simulink model "rfsoc4x2_ospfb_128"  (R2021a)
settings: Solver=VariableStepAuto  StartTime=0.0  StopTime=2048  RelTol=1e-3
undefined symbols (not defined in the file): pfb_coeff_gen_calc
libraries: xbsIndex_r4 x37092, casper_library_delays x737, casper_library_misc x68, xps_library x1
(part 32 of 339)

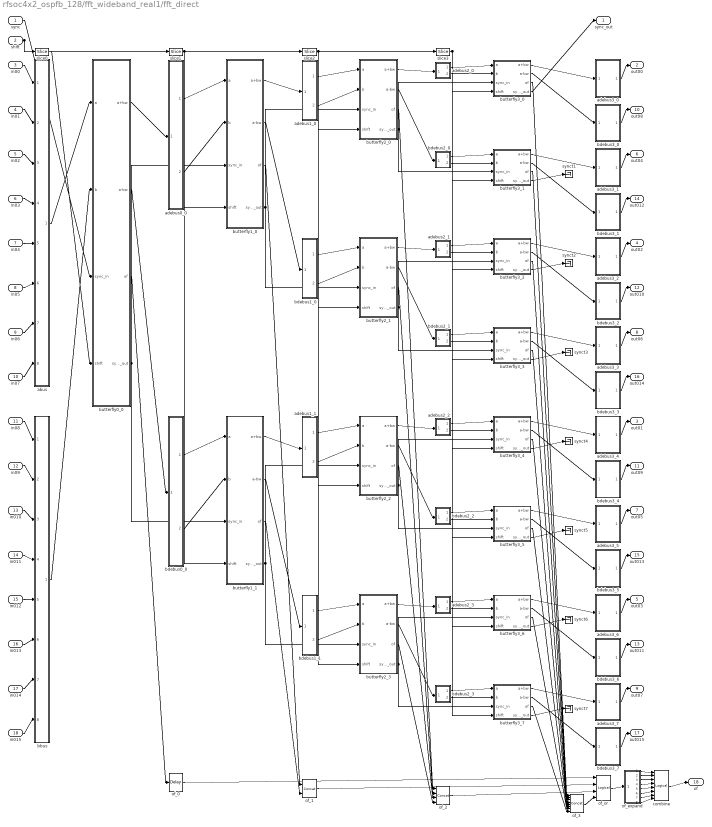
== system rfsoc4x2_ospfb_128/fft_wideband_real1/fft_direct ==
  sync : Inport
  shift : Inport  Port=2
  in00 : Inport  Port=3
  in01 : Inport  Port=4
  in02 : Inport  Port=5
  in03 : Inport  Port=6
  in04 : Inport  Port=7
  in05 : Inport  Port=8
  in06 : Inport  Port=9
  in07 : Inport  Port=10
  in08 : Inport  Port=11
  in09 : Inport  Port=12
  in010 : Inport  Port=13
  in011 : Inport  Port=14
  in012 : Inport  Port=15
  in013 : Inport  Port=16
  in014 : Inport  Port=17
  in015 : Inport  Port=18
  abus : Subsystem  AncestorBlock=casper_library_flow_control/bus_create  mask(bus_create){inputNum=8}
      mask prompts: inputNum "Number of inputs:"
      mask init:
      | bus_create_init(gcb,...
      |     'inputNum', inputNum);
  adebus0_0 : Subsystem  AncestorBlock=casper_library_flow_control/bus_expand  mask(bus_expand){mode=divisions of equal size, outputNum=2, outputWidth=[144 144], outputBinaryPt=[0 0], outputArithmeticType=[0 0], show_format=off, outputToWorkspace=off, variablePrefix=out, outputToModelAsWell=on}
      mask prompts: outputNum "Number of outputs:"; outputWidth "Output width:"; outputBinaryPt "Output binary point position:"; outputArithmeticType "Output arithmetic type (ufix=0, fix=1, bool=2):"; show_format "Print format string?"; outputToWorkspace "Output to workspace?"; variablePrefix "Variable name prefix:"; outputToModelAsWell "Output to model as well?"
      mask help:
      | Expands a 'bus' made using a bus_create or Xilinx
      | concat block.
      | The input will be divided into the specified number
      | of outputs with the specified arithmetic types.
      | Divisions are made from most significant bit.
      mask init: same as rfsoc4x2_ospfb_128/bus_expand1
      settings: AttributesFormatString=2 outputs
      mask TypeOptions mode: divisions of equal size | divisions of arbitrary size
      mask Callback mode: %bus_expand_callback();
      mask Callback outputWidth: %bus_expand_callback();
      mask Callback outputToWorkspace: %bus_expand_callback();
  adebus1_0 : Subsystem  AncestorBlock=casper_library_flow_control/bus_expand  mask(bus_expand){mode=divisions of equal size, outputNum=2, outputWidth=[72 72], outputBinaryPt=[0 0], outputArithmeticType=[0 0], show_format=off, outputToWorkspace=off, variablePrefix=out, outputToModelAsWell=on}
      mask prompts: outputNum "Number of outputs:"; outputWidth "Output width:"; outputBinaryPt "Output binary point position:"; outputArithmeticType "Output arithmetic type (ufix=0, fix=1, bool=2):"; show_format "Print format string?"; outputToWorkspace "Output to workspace?"; variablePrefix "Variable name prefix:"; outputToModelAsWell "Output to model as well?"
      mask help:
      | Expands a 'bus' made using a bus_create or Xilinx
      | concat block.
      | The input will be divided into the specified number
      | of outputs with the specified arithmetic types.
      | Divisions are made from most significant bit.
      mask init: same as rfsoc4x2_ospfb_128/bus_expand1
      settings: AttributesFormatString=2 outputs
      mask TypeOptions mode: divisions of equal size | divisions of arbitrary size
      mask Callback mode: %bus_expand_callback();
      mask Callback outputWidth: %bus_expand_callback();
      mask Callback outputToWorkspace: %bus_expand_callback();
  adebus1_1 : Subsystem  AncestorBlock=casper_library_flow_control/bus_expand  mask(bus_expand){mode=divisions of equal size, outputNum=2, outputWidth=[72 72], outputBinaryPt=[0 0], outputArithmeticType=[0 0], show_format=off, outputToWorkspace=off, variablePrefix=out, outputToModelAsWell=on}
      mask prompts: outputNum "Number of outputs:"; outputWidth "Output width:"; outputBinaryPt "Output binary point position:"; outputArithmeticType "Output arithmetic type (ufix=0, fix=1, bool=2):"; show_format "Print format string?"; outputToWorkspace "Output to workspace?"; variablePrefix "Variable name prefix:"; outputToModelAsWell "Output to model as well?"
      mask help:
      | Expands a 'bus' made using a bus_create or Xilinx
      | concat block.
      | The input will be divided into the specified number
      | of outputs with the specified arithmetic types.
      | Divisions are made from most significant bit.
      mask init: same as rfsoc4x2_ospfb_128/bus_expand1
      settings: AttributesFormatString=2 outputs
      mask TypeOptions mode: divisions of equal size | divisions of arbitrary size
      mask Callback mode: %bus_expand_callback();
      mask Callback outputWidth: %bus_expand_callback();
      mask Callback outputToWorkspace: %bus_expand_callback();
  adebus2_0 : Subsystem  AncestorBlock=casper_library_flow_control/bus_expand  mask(bus_expand){mode=divisions of equal size, outputNum=2, outputWidth=[36 36], outputBinaryPt=[0 0], outputArithmeticType=[0 0], show_format=off, outputToWorkspace=off, variablePrefix=out, outputToModelAsWell=on}
      mask prompts: outputNum "Number of outputs:"; outputWidth "Output width:"; outputBinaryPt "Output binary point position:"; outputArithmeticType "Output arithmetic type (ufix=0, fix=1, bool=2):"; show_format "Print format string?"; outputToWorkspace "Output to workspace?"; variablePrefix "Variable name prefix:"; outputToModelAsWell "Output to model as well?"
      mask help:
      | Expands a 'bus' made using a bus_create or Xilinx
      | concat block.
      | The input will be divided into the specified number
      | of outputs with the specified arithmetic types.
      | Divisions are made from most significant bit.
      mask init: same as rfsoc4x2_ospfb_128/bus_expand1
      settings: AttributesFormatString=2 outputs
      mask TypeOptions mode: divisions of equal size | divisions of arbitrary size
      mask Callback mode: %bus_expand_callback();
      mask Callback outputWidth: %bus_expand_callback();
      mask Callback outputToWorkspace: %bus_expand_callback();
  adebus2_1 : Subsystem  AncestorBlock=casper_library_flow_control/bus_expand  mask(bus_expand){mode=divisions of equal size, outputNum=2, outputWidth=[36 36], outputBinaryPt=[0 0], outputArithmeticType=[0 0], show_format=off, outputToWorkspace=off, variablePrefix=out, outputToModelAsWell=on}
      mask prompts: outputNum "Number of outputs:"; outputWidth "Output width:"; outputBinaryPt "Output binary point position:"; outputArithmeticType "Output arithmetic type (ufix=0, fix=1, bool=2):"; show_format "Print format string?"; outputToWorkspace "Output to workspace?"; variablePrefix "Variable name prefix:"; outputToModelAsWell "Output to model as well?"
      mask help:
      | Expands a 'bus' made using a bus_create or Xilinx
      | concat block.
      | The input will be divided into the specified number
      | of outputs with the specified arithmetic types.
      | Divisions are made from most significant bit.
      mask init: same as rfsoc4x2_ospfb_128/bus_expand1
      settings: AttributesFormatString=2 outputs
      mask TypeOptions mode: divisions of equal size | divisions of arbitrary size
      mask Callback mode: %bus_expand_callback();
      mask Callback outputWidth: %bus_expand_callback();
      mask Callback outputToWorkspace: %bus_expand_callback();
  adebus2_2 : Subsystem  AncestorBlock=casper_library_flow_control/bus_expand  mask(bus_expand){mode=divisions of equal size, outputNum=2, outputWidth=[36 36], outputBinaryPt=[0 0], outputArithmeticType=[0 0], show_format=off, outputToWorkspace=off, variablePrefix=out, outputToModelAsWell=on}
      mask prompts: outputNum "Number of outputs:"; outputWidth "Output width:"; outputBinaryPt "Output binary point position:"; outputArithmeticType "Output arithmetic type (ufix=0, fix=1, bool=2):"; show_format "Print format string?"; outputToWorkspace "Output to workspace?"; variablePrefix "Variable name prefix:"; outputToModelAsWell "Output to model as well?"
      mask help:
      | Expands a 'bus' made using a bus_create or Xilinx
      | concat block.
      | The input will be divided into the specified number
      | of outputs with the specified arithmetic types.
      | Divisions are made from most significant bit.
      mask init: same as rfsoc4x2_ospfb_128/bus_expand1
      settings: AttributesFormatString=2 outputs
      mask TypeOptions mode: divisions of equal size | divisions of arbitrary size
      mask Callback mode: %bus_expand_callback();
      mask Callback outputWidth: %bus_expand_callback();
      mask Callback outputToWorkspace: %bus_expand_callback();
  adebus2_3 : Subsystem  AncestorBlock=casper_library_flow_control/bus_expand  mask(bus_expand){mode=divisions of equal size, outputNum=2, outputWidth=[36 36], outputBinaryPt=[0 0], outputArithmeticType=[0 0], show_format=off, outputToWorkspace=off, variablePrefix=out, outputToModelAsWell=on}
      mask prompts: outputNum "Number of outputs:"; outputWidth "Output width:"; outputBinaryPt "Output binary point position:"; outputArithmeticType "Output arithmetic type (ufix=0, fix=1, bool=2):"; show_format "Print format string?"; outputToWorkspace "Output to workspace?"; variablePrefix "Variable name prefix:"; outputToModelAsWell "Output to model as well?"
      mask help:
      | Expands a 'bus' made using a bus_create or Xilinx
      | concat block.
      | The input will be divided into the specified number
      | of outputs with the specified arithmetic types.
      | Divisions are made from most significant bit.
      mask init: same as rfsoc4x2_ospfb_128/bus_expand1
      settings: AttributesFormatString=2 outputs
      mask TypeOptions mode: divisions of equal size | divisions of arbitrary size
      mask Callback mode: %bus_expand_callback();
      mask Callback outputWidth: %bus_expand_callback();
      mask Callback outputToWorkspace: %bus_expand_callback();
  adebus3_0 : Subsystem  AncestorBlock=casper_library_flow_control/bus_expand  mask(bus_expand){mode=divisions of equal size, outputNum=1, outputWidth=36, outputBinaryPt=0, outputArithmeticType=0, show_format=off, outputToWorkspace=off, variablePrefix=out, outputToModelAsWell=on}
      mask prompts: outputNum "Number of outputs:"; outputWidth "Output width:"; outputBinaryPt "Output binary point position:"; outputArithmeticType "Output arithmetic type (ufix=0, fix=1, bool=2):"; show_format "Print format string?"; outputToWorkspace "Output to workspace?"; variablePrefix "Variable name prefix:"; outputToModelAsWell "Output to model as well?"
      mask help:
      | Expands a 'bus' made using a bus_create or Xilinx
      | concat block.
      | The input will be divided into the specified number
      | of outputs with the specified arithmetic types.
      | Divisions are made from most significant bit.
      mask init: same as rfsoc4x2_ospfb_128/bus_expand1
      settings: AttributesFormatString=1 outputs
      mask TypeOptions mode: divisions of equal size | divisions of arbitrary size
      mask Callback mode: %bus_expand_callback();
      mask Callback outputWidth: %bus_expand_callback();
      mask Callback outputToWorkspace: %bus_expand_callback();
  adebus3_1 : Subsystem  AncestorBlock=casper_library_flow_control/bus_expand  mask(bus_expand){mode=divisions of equal size, outputNum=1, outputWidth=36, outputBinaryPt=0, outputArithmeticType=0, show_format=off, outputToWorkspace=off, variablePrefix=out, outputToModelAsWell=on}
      mask prompts: outputNum "Number of outputs:"; outputWidth "Output width:"; outputBinaryPt "Output binary point position:"; outputArithmeticType "Output arithmetic type (ufix=0, fix=1, bool=2):"; show_format "Print format string?"; outputToWorkspace "Output to workspace?"; variablePrefix "Variable name prefix:"; outputToModelAsWell "Output to model as well?"
      mask help:
      | Expands a 'bus' made using a bus_create or Xilinx
      | concat block.
      | The input will be divided into the specified number
      | of outputs with the specified arithmetic types.
      | Divisions are made from most significant bit.
      mask init: same as rfsoc4x2_ospfb_128/bus_expand1
      settings: AttributesFormatString=1 outputs
      mask TypeOptions mode: divisions of equal size | divisions of arbitrary size
      mask Callback mode: %bus_expand_callback();
      mask Callback outputWidth: %bus_expand_callback();
      mask Callback outputToWorkspace: %bus_expand_callback();
  adebus3_2 : Subsystem  AncestorBlock=casper_library_flow_control/bus_expand  mask(bus_expand){mode=divisions of equal size, outputNum=1, outputWidth=36, outputBinaryPt=0, outputArithmeticType=0, show_format=off, outputToWorkspace=off, variablePrefix=out, outputToModelAsWell=on}
      mask prompts: outputNum "Number of outputs:"; outputWidth "Output width:"; outputBinaryPt "Output binary point position:"; outputArithmeticType "Output arithmetic type (ufix=0, fix=1, bool=2):"; show_format "Print format string?"; outputToWorkspace "Output to workspace?"; variablePrefix "Variable name prefix:"; outputToModelAsWell "Output to model as well?"
      mask help:
      | Expands a 'bus' made using a bus_create or Xilinx
      | concat block.
      | The input will be divided into the specified number
      | of outputs with the specified arithmetic types.
      | Divisions are made from most significant bit.
      mask init: same as rfsoc4x2_ospfb_128/bus_expand1
      settings: AttributesFormatString=1 outputs
      mask TypeOptions mode: divisions of equal size | divisions of arbitrary size
      mask Callback mode: %bus_expand_callback();
      mask Callback outputWidth: %bus_expand_callback();
      mask Callback outputToWorkspace: %bus_expand_callback();
  adebus3_3 : Subsystem  AncestorBlock=casper_library_flow_control/bus_expand  mask(bus_expand){mode=divisions of equal size, outputNum=1, outputWidth=36, outputBinaryPt=0, outputArithmeticType=0, show_format=off, outputToWorkspace=off, variablePrefix=out, outputToModelAsWell=on}
      mask prompts: outputNum "Number of outputs:"; outputWidth "Output width:"; outputBinaryPt "Output binary point position:"; outputArithmeticType "Output arithmetic type (ufix=0, fix=1, bool=2):"; show_format "Print format string?"; outputToWorkspace "Output to workspace?"; variablePrefix "Variable name prefix:"; outputToModelAsWell "Output to model as well?"
      mask help:
      | Expands a 'bus' made using a bus_create or Xilinx
      | concat block.
      | The input will be divided into the specified number
      | of outputs with the specified arithmetic types.
      | Divisions are made from most significant bit.
      mask init: same as rfsoc4x2_ospfb_128/bus_expand1
      settings: AttributesFormatString=1 outputs
      mask TypeOptions mode: divisions of equal size | divisions of arbitrary size
      mask Callback mode: %bus_expand_callback();
      mask Callback outputWidth: %bus_expand_callback();
      mask Callback outputToWorkspace: %bus_expand_callback();
  adebus3_4 : Subsystem  AncestorBlock=casper_library_flow_control/bus_expand  mask(bus_expand){mode=divisions of equal size, outputNum=1, outputWidth=36, outputBinaryPt=0, outputArithmeticType=0, show_format=off, outputToWorkspace=off, variablePrefix=out, outputToModelAsWell=on}
      mask prompts: outputNum "Number of outputs:"; outputWidth "Output width:"; outputBinaryPt "Output binary point position:"; outputArithmeticType "Output arithmetic type (ufix=0, fix=1, bool=2):"; show_format "Print format string?"; outputToWorkspace "Output to workspace?"; variablePrefix "Variable name prefix:"; outputToModelAsWell "Output to model as well?"
      mask help:
      | Expands a 'bus' made using a bus_create or Xilinx
      | concat block.
      | The input will be divided into the specified number
      | of outputs with the specified arithmetic types.
      | Divisions are made from most significant bit.
      mask init: same as rfsoc4x2_ospfb_128/bus_expand1
      settings: AttributesFormatString=1 outputs
      mask TypeOptions mode: divisions of equal size | divisions of arbitrary size
      mask Callback mode: %bus_expand_callback();
      mask Callback outputWidth: %bus_expand_callback();
      mask Callback outputToWorkspace: %bus_expand_callback();
  adebus3_5 : Subsystem  AncestorBlock=casper_library_flow_control/bus_expand  mask(bus_expand){mode=divisions of equal size, outputNum=1, outputWidth=36, outputBinaryPt=0, outputArithmeticType=0, show_format=off, outputToWorkspace=off, variablePrefix=out, outputToModelAsWell=on}
      mask prompts: outputNum "Number of outputs:"; outputWidth "Output width:"; outputBinaryPt "Output binary point position:"; outputArithmeticType "Output arithmetic type (ufix=0, fix=1, bool=2):"; show_format "Print format string?"; outputToWorkspace "Output to workspace?"; variablePrefix "Variable name prefix:"; outputToModelAsWell "Output to model as well?"
      mask help:
      | Expands a 'bus' made using a bus_create or Xilinx
      | concat block.
      | The input will be divided into the specified number
      | of outputs with the specified arithmetic types.
      | Divisions are made from most significant bit.
      mask init: same as rfsoc4x2_ospfb_128/bus_expand1
      settings: AttributesFormatString=1 outputs
      mask TypeOptions mode: divisions of equal size | divisions of arbitrary size
      mask Callback mode: %bus_expand_callback();
      mask Callback outputWidth: %bus_expand_callback();
      mask Callback outputToWorkspace: %bus_expand_callback();
  adebus3_6 : Subsystem  AncestorBlock=casper_library_flow_control/bus_expand  mask(bus_expand){mode=divisions of equal size, outputNum=1, outputWidth=36, outputBinaryPt=0, outputArithmeticType=0, show_format=off, outputToWorkspace=off, variablePrefix=out, outputToModelAsWell=on}
      mask prompts: outputNum "Number of outputs:"; outputWidth "Output width:"; outputBinaryPt "Output binary point position:"; outputArithmeticType "Output arithmetic type (ufix=0, fix=1, bool=2):"; show_format "Print format string?"; outputToWorkspace "Output to workspace?"; variablePrefix "Variable name prefix:"; outputToModelAsWell "Output to model as well?"
      mask help:
      | Expands a 'bus' made using a bus_create or Xilinx
      | concat block.
      | The input will be divided into the specified number
      | of outputs with the specified arithmetic types.
      | Divisions are made from most significant bit.
      mask init: same as rfsoc4x2_ospfb_128/bus_expand1
      settings: AttributesFormatString=1 outputs
      mask TypeOptions mode: divisions of equal size | divisions of arbitrary size
      mask Callback mode: %bus_expand_callback();
      mask Callback outputWidth: %bus_expand_callback();
      mask Callback outputToWorkspace: %bus_expand_callback();
  adebus3_7 : Subsystem  AncestorBlock=casper_library_flow_control/bus_expand  mask(bus_expand){mode=divisions of equal size, outputNum=1, outputWidth=36, outputBinaryPt=0, outputArithmeticType=0, show_format=off, outputToWorkspace=off, variablePrefix=out, outputToModelAsWell=on}
      mask prompts: outputNum "Number of outputs:"; outputWidth "Output width:"; outputBinaryPt "Output binary point position:"; outputArithmeticType "Output arithmetic type (ufix=0, fix=1, bool=2):"; show_format "Print format string?"; outputToWorkspace "Output to workspace?"; variablePrefix "Variable name prefix:"; outputToModelAsWell "Output to model as well?"
      mask help:
      | Expands a 'bus' made using a bus_create or Xilinx
      | concat block.
      | The input will be divided into the specified number
      | of outputs with the specified arithmetic types.
      | Divisions are made from most significant bit.
      mask init: same as rfsoc4x2_ospfb_128/bus_expand1
      settings: AttributesFormatString=1 outputs
      mask TypeOptions mode: divisions of equal size | divisions of arbitrary size
      mask Callback mode: %bus_expand_callback();
      mask Callback outputWidth: %bus_expand_callback();
      mask Callback outputToWorkspace: %bus_expand_callback();
  bbus : Subsystem  AncestorBlock=casper_library_flow_control/bus_create  mask(bus_create){inputNum=8}
      mask prompts: inputNum "Number of inputs:"
      mask init:
      | bus_create_init(gcb,...
      |     'inputNum', inputNum);
  bdebus0_0 : Subsystem  AncestorBlock=casper_library_flow_control/bus_expand  mask(bus_expand){mode=divisions of equal size, outputNum=2, outputWidth=[144 144], outputBinaryPt=[0 0], outputArithmeticType=[0 0], show_format=off, outputToWorkspace=off, variablePrefix=out, outputToModelAsWell=on}
      mask prompts: outputNum "Number of outputs:"; outputWidth "Output width:"; outputBinaryPt "Output binary point position:"; outputArithmeticType "Output arithmetic type (ufix=0, fix=1, bool=2):"; show_format "Print format string?"; outputToWorkspace "Output to workspace?"; variablePrefix "Variable name prefix:"; outputToModelAsWell "Output to model as well?"
      mask help:
      | Expands a 'bus' made using a bus_create or Xilinx
      | concat block.
      | The input will be divided into the specified number
      | of outputs with the specified arithmetic types.
      | Divisions are made from most significant bit.
      mask init: same as rfsoc4x2_ospfb_128/bus_expand1
      settings: AttributesFormatString=2 outputs
      mask TypeOptions mode: divisions of equal size | divisions of arbitrary size
      mask Callback mode: %bus_expand_callback();
      mask Callback outputWidth: %bus_expand_callback();
      mask Callback outputToWorkspace: %bus_expand_callback();
  bdebus1_0 : Subsystem  AncestorBlock=casper_library_flow_control/bus_expand  mask(bus_expand){mode=divisions of equal size, outputNum=2, outputWidth=[72 72], outputBinaryPt=[0 0], outputArithmeticType=[0 0], show_format=off, outputToWorkspace=off, variablePrefix=out, outputToModelAsWell=on}
      mask prompts: outputNum "Number of outputs:"; outputWidth "Output width:"; outputBinaryPt "Output binary point position:"; outputArithmeticType "Output arithmetic type (ufix=0, fix=1, bool=2):"; show_format "Print format string?"; outputToWorkspace "Output to workspace?"; variablePrefix "Variable name prefix:"; outputToModelAsWell "Output to model as well?"
      mask help:
      | Expands a 'bus' made using a bus_create or Xilinx
      | concat block.
      | The input will be divided into the specified number
      | of outputs with the specified arithmetic types.
      | Divisions are made from most significant bit.
      mask init: same as rfsoc4x2_ospfb_128/bus_expand1
      settings: AttributesFormatString=2 outputs
      mask TypeOptions mode: divisions of equal size | divisions of arbitrary size
      mask Callback mode: %bus_expand_callback();
      mask Callback outputWidth: %bus_expand_callback();
      mask Callback outputToWorkspace: %bus_expand_callback();
  bdebus1_1 : Subsystem  AncestorBlock=casper_library_flow_control/bus_expand  mask(bus_expand){mode=divisions of equal size, outputNum=2, outputWidth=[72 72], outputBinaryPt=[0 0], outputArithmeticType=[0 0], show_format=off, outputToWorkspace=off, variablePrefix=out, outputToModelAsWell=on}
      mask prompts: outputNum "Number of outputs:"; outputWidth "Output width:"; outputBinaryPt "Output binary point position:"; outputArithmeticType "Output arithmetic type (ufix=0, fix=1, bool=2):"; show_format "Print format string?"; outputToWorkspace "Output to workspace?"; variablePrefix "Variable name prefix:"; outputToModelAsWell "Output to model as well?"
      mask help:
      | Expands a 'bus' made using a bus_create or Xilinx
      | concat block.
      | The input will be divided into the specified number
      | of outputs with the specified arithmetic types.
      | Divisions are made from most significant bit.
      mask init: same as rfsoc4x2_ospfb_128/bus_expand1
      settings: AttributesFormatString=2 outputs
      mask TypeOptions mode: divisions of equal size | divisions of arbitrary size
      mask Callback mode: %bus_expand_callback();
      mask Callback outputWidth: %bus_expand_callback();
      mask Callback outputToWorkspace: %bus_expand_callback();
  bdebus2_0 : Subsystem  AncestorBlock=casper_library_flow_control/bus_expand  mask(bus_expand){mode=divisions of equal size, outputNum=2, outputWidth=[36 36], outputBinaryPt=[0 0], outputArithmeticType=[0 0], show_format=off, outputToWorkspace=off, variablePrefix=out, outputToModelAsWell=on}
      mask prompts: outputNum "Number of outputs:"; outputWidth "Output width:"; outputBinaryPt "Output binary point position:"; outputArithmeticType "Output arithmetic type (ufix=0, fix=1, bool=2):"; show_format "Print format string?"; outputToWorkspace "Output to workspace?"; variablePrefix "Variable name prefix:"; outputToModelAsWell "Output to model as well?"
      mask help:
      | Expands a 'bus' made using a bus_create or Xilinx
      | concat block.
      | The input will be divided into the specified number
      | of outputs with the specified arithmetic types.
      | Divisions are made from most significant bit.
      mask init: same as rfsoc4x2_ospfb_128/bus_expand1
      settings: AttributesFormatString=2 outputs
      mask TypeOptions mode: divisions of equal size | divisions of arbitrary size
      mask Callback mode: %bus_expand_callback();
      mask Callback outputWidth: %bus_expand_callback();
      mask Callback outputToWorkspace: %bus_expand_callback();
  bdebus2_1 : Subsystem  AncestorBlock=casper_library_flow_control/bus_expand  mask(bus_expand){mode=divisions of equal size, outputNum=2, outputWidth=[36 36], outputBinaryPt=[0 0], outputArithmeticType=[0 0], show_format=off, outputToWorkspace=off, variablePrefix=out, outputToModelAsWell=on}
      mask prompts: outputNum "Number of outputs:"; outputWidth "Output width:"; outputBinaryPt "Output binary point position:"; outputArithmeticType "Output arithmetic type (ufix=0, fix=1, bool=2):"; show_format "Print format string?"; outputToWorkspace "Output to workspace?"; variablePrefix "Variable name prefix:"; outputToModelAsWell "Output to model as well?"
      mask help:
      | Expands a 'bus' made using a bus_create or Xilinx
      | concat block.
      | The input will be divided into the specified number
      | of outputs with the specified arithmetic types.
      | Divisions are made from most significant bit.
      mask init: same as rfsoc4x2_ospfb_128/bus_expand1
      settings: AttributesFormatString=2 outputs
      mask TypeOptions mode: divisions of equal size | divisions of arbitrary size
      mask Callback mode: %bus_expand_callback();
      mask Callback outputWidth: %bus_expand_callback();
      mask Callback outputToWorkspace: %bus_expand_callback();
  bdebus2_2 : Subsystem  AncestorBlock=casper_library_flow_control/bus_expand  mask(bus_expand){mode=divisions of equal size, outputNum=2, outputWidth=[36 36], outputBinaryPt=[0 0], outputArithmeticType=[0 0], show_format=off, outputToWorkspace=off, variablePrefix=out, outputToModelAsWell=on}
      mask prompts: outputNum "Number of outputs:"; outputWidth "Output width:"; outputBinaryPt "Output binary point position:"; outputArithmeticType "Output arithmetic type (ufix=0, fix=1, bool=2):"; show_format "Print format string?"; outputToWorkspace "Output to workspace?"; variablePrefix "Variable name prefix:"; outputToModelAsWell "Output to model as well?"
      mask help:
      | Expands a 'bus' made using a bus_create or Xilinx
      | concat block.
      | The input will be divided into the specified number
      | of outputs with the specified arithmetic types.
      | Divisions are made from most significant bit.
      mask init: same as rfsoc4x2_ospfb_128/bus_expand1
      settings: AttributesFormatString=2 outputs
      mask TypeOptions mode: divisions of equal size | divisions of arbitrary size
      mask Callback mode: %bus_expand_callback();
      mask Callback outputWidth: %bus_expand_callback();
      mask Callback outputToWorkspace: %bus_expand_callback();
  bdebus2_3 : Subsystem  AncestorBlock=casper_library_flow_control/bus_expand  mask(bus_expand){mode=divisions of equal size, outputNum=2, outputWidth=[36 36], outputBinaryPt=[0 0], outputArithmeticType=[0 0], show_format=off, outputToWorkspace=off, variablePrefix=out, outputToModelAsWell=on}
      mask prompts: outputNum "Number of outputs:"; outputWidth "Output width:"; outputBinaryPt "Output binary point position:"; outputArithmeticType "Output arithmetic type (ufix=0, fix=1, bool=2):"; show_format "Print format string?"; outputToWorkspace "Output to workspace?"; variablePrefix "Variable name prefix:"; outputToModelAsWell "Output to model as well?"
      mask help:
      | Expands a 'bus' made using a bus_create or Xilinx
      | concat block.
      | The input will be divided into the specified number
      | of outputs with the specified arithmetic types.
      | Divisions are made from most significant bit.
      mask init: same as rfsoc4x2_ospfb_128/bus_expand1
      settings: AttributesFormatString=2 outputs
      mask TypeOptions mode: divisions of equal size | divisions of arbitrary size
      mask Callback mode: %bus_expand_callback();
      mask Callback outputWidth: %bus_expand_callback();
      mask Callback outputToWorkspace: %bus_expand_callback();
  bdebus3_0 : Subsystem  AncestorBlock=casper_library_flow_control/bus_expand  mask(bus_expand){mode=divisions of equal size, outputNum=1, outputWidth=36, outputBinaryPt=0, outputArithmeticType=0, show_format=off, outputToWorkspace=off, variablePrefix=out, outputToModelAsWell=on}
      mask prompts: outputNum "Number of outputs:"; outputWidth "Output width:"; outputBinaryPt "Output binary point position:"; outputArithmeticType "Output arithmetic type (ufix=0, fix=1, bool=2):"; show_format "Print format string?"; outputToWorkspace "Output to workspace?"; variablePrefix "Variable name prefix:"; outputToModelAsWell "Output to model as well?"
      mask help:
      | Expands a 'bus' made using a bus_create or Xilinx
      | concat block.
      | The input will be divided into the specified number
      | of outputs with the specified arithmetic types.
      | Divisions are made from most significant bit.
      mask init: same as rfsoc4x2_ospfb_128/bus_expand1
      settings: AttributesFormatString=1 outputs
      mask TypeOptions mode: divisions of equal size | divisions of arbitrary size
      mask Callback mode: %bus_expand_callback();
      mask Callback outputWidth: %bus_expand_callback();
      mask Callback outputToWorkspace: %bus_expand_callback();
  bdebus3_1 : Subsystem  AncestorBlock=casper_library_flow_control/bus_expand  mask(bus_expand){mode=divisions of equal size, outputNum=1, outputWidth=36, outputBinaryPt=0, outputArithmeticType=0, show_format=off, outputToWorkspace=off, variablePrefix=out, outputToModelAsWell=on}
      mask prompts: outputNum "Number of outputs:"; outputWidth "Output width:"; outputBinaryPt "Output binary point position:"; outputArithmeticType "Output arithmetic type (ufix=0, fix=1, bool=2):"; show_format "Print format string?"; outputToWorkspace "Output to workspace?"; variablePrefix "Variable name prefix:"; outputToModelAsWell "Output to model as well?"
      mask help:
      | Expands a 'bus' made using a bus_create or Xilinx
      | concat block.
      | The input will be divided into the specified number
      | of outputs with the specified arithmetic types.
      | Divisions are made from most significant bit.
      mask init: same as rfsoc4x2_ospfb_128/bus_expand1
      settings: AttributesFormatString=1 outputs
      mask TypeOptions mode: divisions of equal size | divisions of arbitrary size
      mask Callback mode: %bus_expand_callback();
      mask Callback outputWidth: %bus_expand_callback();
      mask Callback outputToWorkspace: %bus_expand_callback();
  bdebus3_2 : Subsystem  AncestorBlock=casper_library_flow_control/bus_expand  mask(bus_expand){mode=divisions of equal size, outputNum=1, outputWidth=36, outputBinaryPt=0, outputArithmeticType=0, show_format=off, outputToWorkspace=off, variablePrefix=out, outputToModelAsWell=on}
      mask prompts: outputNum "Number of outputs:"; outputWidth "Output width:"; outputBinaryPt "Output binary point position:"; outputArithmeticType "Output arithmetic type (ufix=0, fix=1, bool=2):"; show_format "Print format string?"; outputToWorkspace "Output to workspace?"; variablePrefix "Variable name prefix:"; outputToModelAsWell "Output to model as well?"
      mask help:
      | Expands a 'bus' made using a bus_create or Xilinx
      | concat block.
      | The input will be divided into the specified number
      | of outputs with the specified arithmetic types.
      | Divisions are made from most significant bit.
      mask init: same as rfsoc4x2_ospfb_128/bus_expand1
      settings: AttributesFormatString=1 outputs
      mask TypeOptions mode: divisions of equal size | divisions of arbitrary size
      mask Callback mode: %bus_expand_callback();
      mask Callback outputWidth: %bus_expand_callback();
      mask Callback outputToWorkspace: %bus_expand_callback();
  bdebus3_3 : Subsystem  AncestorBlock=casper_library_flow_control/bus_expand  mask(bus_expand){mode=divisions of equal size, outputNum=1, outputWidth=36, outputBinaryPt=0, outputArithmeticType=0, show_format=off, outputToWorkspace=off, variablePrefix=out, outputToModelAsWell=on}
      mask prompts: outputNum "Number of outputs:"; outputWidth "Output width:"; outputBinaryPt "Output binary point position:"; outputArithmeticType "Output arithmetic type (ufix=0, fix=1, bool=2):"; show_format "Print format string?"; outputToWorkspace "Output to workspace?"; variablePrefix "Variable name prefix:"; outputToModelAsWell "Output to model as well?"
      mask help:
      | Expands a 'bus' made using a bus_create or Xilinx
      | concat block.
      | The input will be divided into the specified number
      | of outputs with the specified arithmetic types.
      | Divisions are made from most significant bit.
      mask init: same as rfsoc4x2_ospfb_128/bus_expand1
      settings: AttributesFormatString=1 outputs
      mask TypeOptions mode: divisions of equal size | divisions of arbitrary size
      mask Callback mode: %bus_expand_callback();
      mask Callback outputWidth: %bus_expand_callback();
      mask Callback outputToWorkspace: %bus_expand_callback();
  bdebus3_4 : Subsystem  AncestorBlock=casper_library_flow_control/bus_expand  mask(bus_expand){mode=divisions of equal size, outputNum=1, outputWidth=36, outputBinaryPt=0, outputArithmeticType=0, show_format=off, outputToWorkspace=off, variablePrefix=out, outputToModelAsWell=on}
      mask prompts: outputNum "Number of outputs:"; outputWidth "Output width:"; outputBinaryPt "Output binary point position:"; outputArithmeticType "Output arithmetic type (ufix=0, fix=1, bool=2):"; show_format "Print format string?"; outputToWorkspace "Output to workspace?"; variablePrefix "Variable name prefix:"; outputToModelAsWell "Output to model as well?"
      mask help:
      | Expands a 'bus' made using a bus_create or Xilinx
      | concat block.
      | The input will be divided into the specified number
      | of outputs with the specified arithmetic types.
      | Divisions are made from most significant bit.
      mask init: same as rfsoc4x2_ospfb_128/bus_expand1
      settings: AttributesFormatString=1 outputs
      mask TypeOptions mode: divisions of equal size | divisions of arbitrary size
      mask Callback mode: %bus_expand_callback();
      mask Callback outputWidth: %bus_expand_callback();
      mask Callback outputToWorkspace: %bus_expand_callback();
  bdebus3_5 : Subsystem  AncestorBlock=casper_library_flow_control/bus_expand  mask(bus_expand){mode=divisions of equal size, outputNum=1, outputWidth=36, outputBinaryPt=0, outputArithmeticType=0, show_format=off, outputToWorkspace=off, variablePrefix=out, outputToModelAsWell=on}
      mask prompts: outputNum "Number of outputs:"; outputWidth "Output width:"; outputBinaryPt "Output binary point position:"; outputArithmeticType "Output arithmetic type (ufix=0, fix=1, bool=2):"; show_format "Print format string?"; outputToWorkspace "Output to workspace?"; variablePrefix "Variable name prefix:"; outputToModelAsWell "Output to model as well?"
      mask help:
      | Expands a 'bus' made using a bus_create or Xilinx
      | concat block.
      | The input will be divided into the specified number
      | of outputs with the specified arithmetic types.
      | Divisions are made from most significant bit.
      mask init: same as rfsoc4x2_ospfb_128/bus_expand1
      settings: AttributesFormatString=1 outputs
      mask TypeOptions mode: divisions of equal size | divisions of arbitrary size
      mask Callback mode: %bus_expand_callback();
      mask Callback outputWidth: %bus_expand_callback();
      mask Callback outputToWorkspace: %bus_expand_callback();
  bdebus3_6 : Subsystem  AncestorBlock=casper_library_flow_control/bus_expand  mask(bus_expand){mode=divisions of equal size, outputNum=1, outputWidth=36, outputBinaryPt=0, outputArithmeticType=0, show_format=off, outputToWorkspace=off, variablePrefix=out, outputToModelAsWell=on}
      mask prompts: outputNum "Number of outputs:"; outputWidth "Output width:"; outputBinaryPt "Output binary point position:"; outputArithmeticType "Output arithmetic type (ufix=0, fix=1, bool=2):"; show_format "Print format string?"; outputToWorkspace "Output to workspace?"; variablePrefix "Variable name prefix:"; outputToModelAsWell "Output to model as well?"
      mask help:
      | Expands a 'bus' made using a bus_create or Xilinx
      | concat block.
      | The input will be divided into the specified number
      | of outputs with the specified arithmetic types.
      | Divisions are made from most significant bit.
      mask init: same as rfsoc4x2_ospfb_128/bus_expand1
      settings: AttributesFormatString=1 outputs
      mask TypeOptions mode: divisions of equal size | divisions of arbitrary size
      mask Callback mode: %bus_expand_callback();
      mask Callback outputWidth: %bus_expand_callback();
      mask Callback outputToWorkspace: %bus_expand_callback();
  bdebus3_7 : Subsystem  AncestorBlock=casper_library_flow_control/bus_expand  mask(bus_expand){mode=divisions of equal size, outputNum=1, outputWidth=36, outputBinaryPt=0, outputArithmeticType=0, show_format=off, outputToWorkspace=off, variablePrefix=out, outputToModelAsWell=on}
      mask prompts: outputNum "Number of outputs:"; outputWidth "Output width:"; outputBinaryPt "Output binary point position:"; outputArithmeticType "Output arithmetic type (ufix=0, fix=1, bool=2):"; show_format "Print format string?"; outputToWorkspace "Output to workspace?"; variablePrefix "Variable name prefix:"; outputToModelAsWell "Output to model as well?"
      mask help:
      | Expands a 'bus' made using a bus_create or Xilinx
      | concat block.
      | The input will be divided into the specified number
      | of outputs with the specified arithmetic types.
      | Divisions are made from most significant bit.
      mask init: same as rfsoc4x2_ospfb_128/bus_expand1
      settings: AttributesFormatString=1 outputs
      mask TypeOptions mode: divisions of equal size | divisions of arbitrary size
      mask Callback mode: %bus_expand_callback();
      mask Callback outputWidth: %bus_expand_callback();
      mask Callback outputToWorkspace: %bus_expand_callback();
  butterfly0_0 : Subsystem  AncestorBlock=casper_library_ffts/butterfly_direct  mask(butterfly_direct){n_inputs=8, biplex=off, FFTSize=8, Coeffs=[ 0 8 4 12 2 10 6 14 1 9 5 13 3 11 7 15], StepPeriod=0, coeff_bit_width=18, input_bit_width=18, bin_pt_in=17, downshift=off, async=off, floating_point=off, float_type=single, exp_width=8, frac_width=24, add_latency=1, mult_latency=3, bram_latency=3, conv_latency=3, add_pipe_latency=0, mult_pipe_latency=0, quantization=Round  (unbiased: +/- Inf), overflow=Wrap, coeffs_bit_limit=8, coeff_sharing=off, coeff_decimation=off, coeff_generation=off, cal_bits=1, n_bits_rotation=25, max_fanout=4, use_hdl=on, use_embedded=off, bitgrowth=off, hardcode_shifts=off, dsp48_adders=off}
      mask prompts: n_inputs "number inputs"; biplex "Used in biplex FFT"; FFTSize "Size of FFT: (2^? pts)"; Coeffs "Coefficients: (0 to 2^(FFTSize-1)-1)"; StepPeriod "Coefficient Step Period: (2^?)"; coeff_bit_width "Coefficient Bit Width"; input_bit_width "Input Bit Width"; bin_pt_in "Input binary point"; async "asynchronous operation"; floating_point "floating point"; float_type "float type"; exp_width "exponent width"; frac_width "fraction width"; add_latency "Add Latency"; mult_latency "Mult Latency"; bram_latency "BRAM Latency"; conv_latency "Convert latency"; add_pipe_latency "Add Pipeline Latency"; mult_pipe_latency "Mult Pipeline Latency"; quantization "Quantization Behavior"; overflow "Overflow Behavior"; coeffs_bit_limit "Number bits above which to store stage's coefficients in BRAM (2^? bits)"; coeff_sharing "BRAM sharing in coeff storage"; coeff_decimation "Store a fraction of coeff factors where useful"; coeff_generation "Generate coeffs with multipliers where useful"; cal_bits "Number calibration locations when generating coeffs (2^?)"; n_bits_rotation "Feedback rotation vector resolution"; max_fanout "Maximum fanout"; use_hdl "Use behavioural HDL for multipliers"; use_embedded "Use embedded multipliers"; bitgrowth "Bit growth instead of shifting"; hardcode_shifts "Hardcode shift schedule"; dsp48_adders "Use DSP48s for adders"
      mask help: FFT internal block.
      mask init: same as rfsoc4x2_ospfb_128/fft2/fft_direct/butterfly0_0
      settings: AttributesFormatString=twiddle_general
      mask Callback floating_point:
      | onoff = get_param(gcb, 'floating_point');
      | if strcmp(onoff,'on')
      |     enable_fixpt = 'off';
      |     set_param_state(gcb, 'float_type', 'on')
      | 
      |     f_type = get_param(gcb, 'float_type');
      |     if strcmp(f_type,'custom')
      |         set_param_state(gcb, 'exp_width', 'on')
      |         set_param_state(gcb, 'frac_width', 'on')
      |     else
      |         set_param_state(gcb, 'exp_width', 'off')
      |         set_param_state(gcb, 'frac_width', 'off')
      |     end
      | 
      | 
      | else
      |     enable_fixpt = 'on';
      |     set_param_state(gcb, 'float_type', 'off')
      |     set_param_state(gcb, 'exp_width', 'off')
      |     set_param_state(gcb, 'frac_width', 'off')
      | end
      | 
      | set_param_state(gcb, 'input_bit_width', enable_fixpt)
      | set_param_state(gcb, 'bin_pt_in', enable_fixpt)
      | set_param_state(gcb, 'coeff_bit_width', enable_fixpt)
      mask TypeOptions float_type: single | custom
      mask Callback float_type:
      | f_type = get_param(gcb, 'float_type');
      | if strcmp(f_type,'custom')
      |     set_param_state(gcb, 'exp_width', 'on')
      |     set_param_state(gcb, 'frac_width', 'on')
      | else
      |     set_param_state(gcb, 'exp_width', 'off')
      |     set_param_state(gcb, 'frac_width', 'off')
      | end
      mask TypeOptions quantization: Truncate | Round  (unbiased: +/- Inf) | Round  (unbiased: Even Values)
      mask TypeOptions overflow: Wrap | Saturate | Error
      mask Callback use_hdl:
      | % make mutually exclusive with use_embedded.
      | 
      | use_hdl = get_param(gcb, 'use_hdl');
      | if strcmp(use_hdl, 'on'),
      |     set_param_state(gcb, 'use_embedded', 'off');
      | else
      |     set_param_state(gcb, 'use_embedded', 'on');
      | end
      mask Callback use_embedded:
      | % make mutually exclusive with use_hdl.
      | 
      | use_hdl = get_param(gcb, 'use_embedded');
      | if strcmp(use_hdl, 'on'),
      |     set_param_state(gcb, 'use_hdl', 'off');
      | else
      |     set_param_state(gcb, 'use_hdl', 'on');
      | end
      mask Callback hardcode_shifts:
      | hardcode_shifts = get_param(gcb, 'hardcode_shifts');
      | set_param_state(gcb, 'downshift', hardcode_shifts);
      mask Callback dsp48_adders: %fft_callback_dsp48_adders(gcb);
      mask DialogControl ParameterTabVar0 Prompt: Basic
      mask DialogControl ParameterTabVar01 Prompt: Latency
      mask DialogControl ParameterTabVar012 Prompt: Implementation
  butterfly1_0 : Subsystem  AncestorBlock=casper_library_ffts/butterfly_direct  mask(butterfly_direct){n_inputs=4, biplex=off, FFTSize=8, Coeffs=[ 0 16 8 24 4 20 12 28 2 18 10 26 6 22 14 30], StepPeriod=0, coeff_bit_width=18, input_bit_width=18, bin_pt_in=17, downshift=off, async=off, floating_point=off, float_type=single, exp_width=8, frac_width=24, add_latency=1, mult_latency=3, bram_latency=3, conv_latency=3, add_pipe_latency=0, mult_pipe_latency=0, quantization=Round  (unbiased: +/- Inf), overflow=Wrap, coeffs_bit_limit=8, coeff_sharing=off, coeff_decimation=off, coeff_generation=off, cal_bits=1, n_bits_rotation=25, max_fanout=4, use_hdl=on, use_embedded=off, bitgrowth=off, hardcode_shifts=off, dsp48_adders=off}
      mask prompts: n_inputs "number inputs"; biplex "Used in biplex FFT"; FFTSize "Size of FFT: (2^? pts)"; Coeffs "Coefficients: (0 to 2^(FFTSize-1)-1)"; StepPeriod "Coefficient Step Period: (2^?)"; coeff_bit_width "Coefficient Bit Width"; input_bit_width "Input Bit Width"; bin_pt_in "Input binary point"; async "asynchronous operation"; floating_point "floating point"; float_type "float type"; exp_width "exponent width"; frac_width "fraction width"; add_latency "Add Latency"; mult_latency "Mult Latency"; bram_latency "BRAM Latency"; conv_latency "Convert latency"; add_pipe_latency "Add Pipeline Latency"; mult_pipe_latency "Mult Pipeline Latency"; quantization "Quantization Behavior"; overflow "Overflow Behavior"; coeffs_bit_limit "Number bits above which to store stage's coefficients in BRAM (2^? bits)"; coeff_sharing "BRAM sharing in coeff storage"; coeff_decimation "Store a fraction of coeff factors where useful"; coeff_generation "Generate coeffs with multipliers where useful"; cal_bits "Number calibration locations when generating coeffs (2^?)"; n_bits_rotation "Feedback rotation vector resolution"; max_fanout "Maximum fanout"; use_hdl "Use behavioural HDL for multipliers"; use_embedded "Use embedded multipliers"; bitgrowth "Bit growth instead of shifting"; hardcode_shifts "Hardcode shift schedule"; dsp48_adders "Use DSP48s for adders"
      mask help: FFT internal block.
      mask init: same as rfsoc4x2_ospfb_128/fft2/fft_direct/butterfly0_0
      settings: AttributesFormatString=twiddle_general
      mask Callback floating_point:
      | onoff = get_param(gcb, 'floating_point');
      | if strcmp(onoff,'on')
      |     enable_fixpt = 'off';
      |     set_param_state(gcb, 'float_type', 'on')
      | 
      |     f_type = get_param(gcb, 'float_type');
      |     if strcmp(f_type,'custom')
      |         set_param_state(gcb, 'exp_width', 'on')
      |         set_param_state(gcb, 'frac_width', 'on')
      |     else
      |         set_param_state(gcb, 'exp_width', 'off')
      |         set_param_state(gcb, 'frac_width', 'off')
      |     end
      | 
      | 
      | else
      |     enable_fixpt = 'on';
      |     set_param_state(gcb, 'float_type', 'off')
      |     set_param_state(gcb, 'exp_width', 'off')
      |     set_param_state(gcb, 'frac_width', 'off')
      | end
      | 
      | set_param_state(gcb, 'input_bit_width', enable_fixpt)
      | set_param_state(gcb, 'bin_pt_in', enable_fixpt)
      | set_param_state(gcb, 'coeff_bit_width', enable_fixpt)
      mask TypeOptions float_type: single | custom
      mask Callback float_type:
      | f_type = get_param(gcb, 'float_type');
      | if strcmp(f_type,'custom')
      |     set_param_state(gcb, 'exp_width', 'on')
      |     set_param_state(gcb, 'frac_width', 'on')
      | else
      |     set_param_state(gcb, 'exp_width', 'off')
      |     set_param_state(gcb, 'frac_width', 'off')
      | end
      mask TypeOptions quantization: Truncate | Round  (unbiased: +/- Inf) | Round  (unbiased: Even Values)
      mask TypeOptions overflow: Wrap | Saturate | Error
      mask Callback use_hdl:
      | % make mutually exclusive with use_embedded.
      | 
      | use_hdl = get_param(gcb, 'use_hdl');
      | if strcmp(use_hdl, 'on'),
      |     set_param_state(gcb, 'use_embedded', 'off');
      | else
      |     set_param_state(gcb, 'use_embedded', 'on');
      | end
      mask Callback use_embedded:
      | % make mutually exclusive with use_hdl.
      | 
      | use_hdl = get_param(gcb, 'use_embedded');
      | if strcmp(use_hdl, 'on'),
      |     set_param_state(gcb, 'use_hdl', 'off');
      | else
      |     set_param_state(gcb, 'use_hdl', 'on');
      | end
      mask Callback hardcode_shifts:
      | hardcode_shifts = get_param(gcb, 'hardcode_shifts');
      | set_param_state(gcb, 'downshift', hardcode_shifts);
      mask Callback dsp48_adders: %fft_callback_dsp48_adders(gcb);
      mask DialogControl ParameterTabVar0 Prompt: Basic
      mask DialogControl ParameterTabVar01 Prompt: Latency
      mask DialogControl ParameterTabVar012 Prompt: Implementation
  butterfly1_1 : Subsystem  AncestorBlock=casper_library_ffts/butterfly_direct  mask(butterfly_direct){n_inputs=4, biplex=off, FFTSize=8, Coeffs=[ 1 17 9 25 5 21 13 29 3 19 11 27 7 23 15 31], StepPeriod=0, coeff_bit_width=18, input_bit_width=18, bin_pt_in=17, downshift=off, async=off, floating_point=off, float_type=single, exp_width=8, frac_width=24, add_latency=1, mult_latency=3, bram_latency=3, conv_latency=3, add_pipe_latency=0, mult_pipe_latency=0, quantization=Round  (unbiased: +/- Inf), overflow=Wrap, coeffs_bit_limit=8, coeff_sharing=off, coeff_decimation=off, coeff_generation=off, cal_bits=1, n_bits_rotation=25, max_fanout=4, use_hdl=on, use_embedded=off, bitgrowth=off, hardcode_shifts=off, dsp48_adders=off}
      mask prompts: n_inputs "number inputs"; biplex "Used in biplex FFT"; FFTSize "Size of FFT: (2^? pts)"; Coeffs "Coefficients: (0 to 2^(FFTSize-1)-1)"; StepPeriod "Coefficient Step Period: (2^?)"; coeff_bit_width "Coefficient Bit Width"; input_bit_width "Input Bit Width"; bin_pt_in "Input binary point"; async "asynchronous operation"; floating_point "floating point"; float_type "float type"; exp_width "exponent width"; frac_width "fraction width"; add_latency "Add Latency"; mult_latency "Mult Latency"; bram_latency "BRAM Latency"; conv_latency "Convert latency"; add_pipe_latency "Add Pipeline Latency"; mult_pipe_latency "Mult Pipeline Latency"; quantization "Quantization Behavior"; overflow "Overflow Behavior"; coeffs_bit_limit "Number bits above which to store stage's coefficients in BRAM (2^? bits)"; coeff_sharing "BRAM sharing in coeff storage"; coeff_decimation "Store a fraction of coeff factors where useful"; coeff_generation "Generate coeffs with multipliers where useful"; cal_bits "Number calibration locations when generating coeffs (2^?)"; n_bits_rotation "Feedback rotation vector resolution"; max_fanout "Maximum fanout"; use_hdl "Use behavioural HDL for multipliers"; use_embedded "Use embedded multipliers"; bitgrowth "Bit growth instead of shifting"; hardcode_shifts "Hardcode shift schedule"; dsp48_adders "Use DSP48s for adders"
      mask help: FFT internal block.
      mask init: same as rfsoc4x2_ospfb_128/fft2/fft_direct/butterfly0_0
      settings: AttributesFormatString=twiddle_general
      mask Callback floating_point:
      | onoff = get_param(gcb, 'floating_point');
      | if strcmp(onoff,'on')
      |     enable_fixpt = 'off';
      |     set_param_state(gcb, 'float_type', 'on')
      | 
      |     f_type = get_param(gcb, 'float_type');
      |     if strcmp(f_type,'custom')
      |         set_param_state(gcb, 'exp_width', 'on')
      |         set_param_state(gcb, 'frac_width', 'on')
      |     else
      |         set_param_state(gcb, 'exp_width', 'off')
      |         set_param_state(gcb, 'frac_width', 'off')
      |     end
      | 
      | 
      | else
      |     enable_fixpt = 'on';
      |     set_param_state(gcb, 'float_type', 'off')
      |     set_param_state(gcb, 'exp_width', 'off')
      |     set_param_state(gcb, 'frac_width', 'off')
      | end
      | 
      | set_param_state(gcb, 'input_bit_width', enable_fixpt)
      | set_param_state(gcb, 'bin_pt_in', enable_fixpt)
      | set_param_state(gcb, 'coeff_bit_width', enable_fixpt)
      mask TypeOptions float_type: single | custom
      mask Callback float_type:
      | f_type = get_param(gcb, 'float_type');
      | if strcmp(f_type,'custom')
      |     set_param_state(gcb, 'exp_width', 'on')
      |     set_param_state(gcb, 'frac_width', 'on')
      | else
      |     set_param_state(gcb, 'exp_width', 'off')
      |     set_param_state(gcb, 'frac_width', 'off')
      | end
      mask TypeOptions quantization: Truncate | Round  (unbiased: +/- Inf) | Round  (unbiased: Even Values)
      mask TypeOptions overflow: Wrap | Saturate | Error
      mask Callback use_hdl:
      | % make mutually exclusive with use_embedded.
      | 
      | use_hdl = get_param(gcb, 'use_hdl');
      | if strcmp(use_hdl, 'on'),
      |     set_param_state(gcb, 'use_embedded', 'off');
      | else
      |     set_param_state(gcb, 'use_embedded', 'on');
      | end
      mask Callback use_embedded:
      | % make mutually exclusive with use_hdl.
      | 
      | use_hdl = get_param(gcb, 'use_embedded');
      | if strcmp(use_hdl, 'on'),
      |     set_param_state(gcb, 'use_hdl', 'off');
      | else
      |     set_param_state(gcb, 'use_hdl', 'on');
      | end
      mask Callback hardcode_shifts:
      | hardcode_shifts = get_param(gcb, 'hardcode_shifts');
      | set_param_state(gcb, 'downshift', hardcode_shifts);
      mask Callback dsp48_adders: %fft_callback_dsp48_adders(gcb);
      mask DialogControl ParameterTabVar0 Prompt: Basic
      mask DialogControl ParameterTabVar01 Prompt: Latency
      mask DialogControl ParameterTabVar012 Prompt: Implementation
  butterfly2_0 : Subsystem  AncestorBlock=casper_library_ffts/butterfly_direct  mask(butterfly_direct){n_inputs=2, biplex=off, FFTSize=8, Coeffs=[ 0 32 16 48 8 40 24 56 4 36 20 52 12 44 28 60], StepPeriod=0, coeff_bit_width=18, input_bit_width=18, bin_pt_in=17, downshift=off, async=off, floating_point=off, float_type=single, exp_width=8, frac_width=24, add_latency=1, mult_latency=3, bram_latency=3, conv_latency=3, add_pipe_latency=0, mult_pipe_latency=0, quantization=Round  (unbiased: +/- Inf), overflow=Wrap, coeffs_bit_limit=8, coeff_sharing=off, coeff_decimation=off, coeff_generation=off, cal_bits=1, n_bits_rotation=25, max_fanout=4, use_hdl=on, use_embedded=off, bitgrowth=off, hardcode_shifts=off, dsp48_adders=off}
      mask prompts: n_inputs "number inputs"; biplex "Used in biplex FFT"; FFTSize "Size of FFT: (2^? pts)"; Coeffs "Coefficients: (0 to 2^(FFTSize-1)-1)"; StepPeriod "Coefficient Step Period: (2^?)"; coeff_bit_width "Coefficient Bit Width"; input_bit_width "Input Bit Width"; bin_pt_in "Input binary point"; async "asynchronous operation"; floating_point "floating point"; float_type "float type"; exp_width "exponent width"; frac_width "fraction width"; add_latency "Add Latency"; mult_latency "Mult Latency"; bram_latency "BRAM Latency"; conv_latency "Convert latency"; add_pipe_latency "Add Pipeline Latency"; mult_pipe_latency "Mult Pipeline Latency"; quantization "Quantization Behavior"; overflow "Overflow Behavior"; coeffs_bit_limit "Number bits above which to store stage's coefficients in BRAM (2^? bits)"; coeff_sharing "BRAM sharing in coeff storage"; coeff_decimation "Store a fraction of coeff factors where useful"; coeff_generation "Generate coeffs with multipliers where useful"; cal_bits "Number calibration locations when generating coeffs (2^?)"; n_bits_rotation "Feedback rotation vector resolution"; max_fanout "Maximum fanout"; use_hdl "Use behavioural HDL for multipliers"; use_embedded "Use embedded multipliers"; bitgrowth "Bit growth instead of shifting"; hardcode_shifts "Hardcode shift schedule"; dsp48_adders "Use DSP48s for adders"
      mask help: FFT internal block.
      mask init: same as rfsoc4x2_ospfb_128/fft2/fft_direct/butterfly0_0
      settings: AttributesFormatString=twiddle_general
      mask Callback floating_point:
      | onoff = get_param(gcb, 'floating_point');
      | if strcmp(onoff,'on')
      |     enable_fixpt = 'off';
      |     set_param_state(gcb, 'float_type', 'on')
      | 
      |     f_type = get_param(gcb, 'float_type');
      |     if strcmp(f_type,'custom')
      |         set_param_state(gcb, 'exp_width', 'on')
      |         set_param_state(gcb, 'frac_width', 'on')
      |     else
      |         set_param_state(gcb, 'exp_width', 'off')
      |         set_param_state(gcb, 'frac_width', 'off')
      |     end
      | 
      | 
      | else
      |     enable_fixpt = 'on';
      |     set_param_state(gcb, 'float_type', 'off')
      |     set_param_state(gcb, 'exp_width', 'off')
      |     set_param_state(gcb, 'frac_width', 'off')
      | end
      | 
      | set_param_state(gcb, 'input_bit_width', enable_fixpt)
      | set_param_state(gcb, 'bin_pt_in', enable_fixpt)
      | set_param_state(gcb, 'coeff_bit_width', enable_fixpt)
      mask TypeOptions float_type: single | custom
      mask Callback float_type:
      | f_type = get_param(gcb, 'float_type');
      | if strcmp(f_type,'custom')
      |     set_param_state(gcb, 'exp_width', 'on')
      |     set_param_state(gcb, 'frac_width', 'on')
      | else
      |     set_param_state(gcb, 'exp_width', 'off')
      |     set_param_state(gcb, 'frac_width', 'off')
      | end
      mask TypeOptions quantization: Truncate | Round  (unbiased: +/- Inf) | Round  (unbiased: Even Values)
      mask TypeOptions overflow: Wrap | Saturate | Error
      mask Callback use_hdl:
      | % make mutually exclusive with use_embedded.
      | 
      | use_hdl = get_param(gcb, 'use_hdl');
      | if strcmp(use_hdl, 'on'),
      |     set_param_state(gcb, 'use_embedded', 'off');
      | else
      |     set_param_state(gcb, 'use_embedded', 'on');
      | end
      mask Callback use_embedded:
      | % make mutually exclusive with use_hdl.
      | 
      | use_hdl = get_param(gcb, 'use_embedded');
      | if strcmp(use_hdl, 'on'),
      |     set_param_state(gcb, 'use_hdl', 'off');
      | else
      |     set_param_state(gcb, 'use_hdl', 'on');
      | end
      mask Callback hardcode_shifts:
      | hardcode_shifts = get_param(gcb, 'hardcode_shifts');
      | set_param_state(gcb, 'downshift', hardcode_shifts);
      mask Callback dsp48_adders: %fft_callback_dsp48_adders(gcb);
      mask DialogControl ParameterTabVar0 Prompt: Basic
      mask DialogControl ParameterTabVar01 Prompt: Latency
      mask DialogControl ParameterTabVar012 Prompt: Implementation
  butterfly2_1 : Subsystem  AncestorBlock=casper_library_ffts/butterfly_direct  mask(butterfly_direct){n_inputs=2, biplex=off, FFTSize=8, Coeffs=[ 1 33 17 49 9 41 25 57 5 37 21 53 13 45 29 61], StepPeriod=0, coeff_bit_width=18, input_bit_width=18, bin_pt_in=17, downshift=off, async=off, floating_point=off, float_type=single, exp_width=8, frac_width=24, add_latency=1, mult_latency=3, bram_latency=3, conv_latency=3, add_pipe_latency=0, mult_pipe_latency=0, quantization=Round  (unbiased: +/- Inf), overflow=Wrap, coeffs_bit_limit=8, coeff_sharing=off, coeff_decimation=off, coeff_generation=off, cal_bits=1, n_bits_rotation=25, max_fanout=4, use_hdl=on, use_embedded=off, bitgrowth=off, hardcode_shifts=off, dsp48_adders=off}
      mask prompts: n_inputs "number inputs"; biplex "Used in biplex FFT"; FFTSize "Size of FFT: (2^? pts)"; Coeffs "Coefficients: (0 to 2^(FFTSize-1)-1)"; StepPeriod "Coefficient Step Period: (2^?)"; coeff_bit_width "Coefficient Bit Width"; input_bit_width "Input Bit Width"; bin_pt_in "Input binary point"; async "asynchronous operation"; floating_point "floating point"; float_type "float type"; exp_width "exponent width"; frac_width "fraction width"; add_latency "Add Latency"; mult_latency "Mult Latency"; bram_latency "BRAM Latency"; conv_latency "Convert latency"; add_pipe_latency "Add Pipeline Latency"; mult_pipe_latency "Mult Pipeline Latency"; quantization "Quantization Behavior"; overflow "Overflow Behavior"; coeffs_bit_limit "Number bits above which to store stage's coefficients in BRAM (2^? bits)"; coeff_sharing "BRAM sharing in coeff storage"; coeff_decimation "Store a fraction of coeff factors where useful"; coeff_generation "Generate coeffs with multipliers where useful"; cal_bits "Number calibration locations when generating coeffs (2^?)"; n_bits_rotation "Feedback rotation vector resolution"; max_fanout "Maximum fanout"; use_hdl "Use behavioural HDL for multipliers"; use_embedded "Use embedded multipliers"; bitgrowth "Bit growth instead of shifting"; hardcode_shifts "Hardcode shift schedule"; dsp48_adders "Use DSP48s for adders"
      mask help: FFT internal block.
      mask init: same as rfsoc4x2_ospfb_128/fft2/fft_direct/butterfly0_0
      settings: AttributesFormatString=twiddle_general
      mask Callback floating_point:
      | onoff = get_param(gcb, 'floating_point');
      | if strcmp(onoff,'on')
      |     enable_fixpt = 'off';
      |     set_param_state(gcb, 'float_type', 'on')
      | 
      |     f_type = get_param(gcb, 'float_type');
      |     if strcmp(f_type,'custom')
      |         set_param_state(gcb, 'exp_width', 'on')
      |         set_param_state(gcb, 'frac_width', 'on')
      |     else
      |         set_param_state(gcb, 'exp_width', 'off')
      |         set_param_state(gcb, 'frac_width', 'off')
      |     end
      | 
      | 
      | else
      |     enable_fixpt = 'on';
      |     set_param_state(gcb, 'float_type', 'off')
      |     set_param_state(gcb, 'exp_width', 'off')
      |     set_param_state(gcb, 'frac_width', 'off')
      | end
      | 
      | set_param_state(gcb, 'input_bit_width', enable_fixpt)
      | set_param_state(gcb, 'bin_pt_in', enable_fixpt)
      | set_param_state(gcb, 'coeff_bit_width', enable_fixpt)
      mask TypeOptions float_type: single | custom
      mask Callback float_type:
      | f_type = get_param(gcb, 'float_type');
      | if strcmp(f_type,'custom')
      |     set_param_state(gcb, 'exp_width', 'on')
      |     set_param_state(gcb, 'frac_width', 'on')
      | else
      |     set_param_state(gcb, 'exp_width', 'off')
      |     set_param_state(gcb, 'frac_width', 'off')
      | end
      mask TypeOptions quantization: Truncate | Round  (unbiased: +/- Inf) | Round  (unbiased: Even Values)
      mask TypeOptions overflow: Wrap | Saturate | Error
      mask Callback use_hdl:
      | % make mutually exclusive with use_embedded.
      | 
      | use_hdl = get_param(gcb, 'use_hdl');
      | if strcmp(use_hdl, 'on'),
      |     set_param_state(gcb, 'use_embedded', 'off');
      | else
      |     set_param_state(gcb, 'use_embedded', 'on');
      | end
      mask Callback use_embedded:
      | % make mutually exclusive with use_hdl.
      | 
      | use_hdl = get_param(gcb, 'use_embedded');
      | if strcmp(use_hdl, 'on'),
      |     set_param_state(gcb, 'use_hdl', 'off');
      | else
      |     set_param_state(gcb, 'use_hdl', 'on');
      | end
      mask Callback hardcode_shifts:
      | hardcode_shifts = get_param(gcb, 'hardcode_shifts');
      | set_param_state(gcb, 'downshift', hardcode_shifts);
      mask Callback dsp48_adders: %fft_callback_dsp48_adders(gcb);
      mask DialogControl ParameterTabVar0 Prompt: Basic
      mask DialogControl ParameterTabVar01 Prompt: Latency
      mask DialogControl ParameterTabVar012 Prompt: Implementation
  butterfly2_2 : Subsystem  AncestorBlock=casper_library_ffts/butterfly_direct  mask(butterfly_direct){n_inputs=2, biplex=off, FFTSize=8, Coeffs=[ 2 34 18 50 10 42 26 58 6 38 22 54 14 46 30 62], StepPeriod=0, coeff_bit_width=18, input_bit_width=18, bin_pt_in=17, downshift=off, async=off, floating_point=off, float_type=single, exp_width=8, frac_width=24, add_latency=1, mult_latency=3, bram_latency=3, conv_latency=3, add_pipe_latency=0, mult_pipe_latency=0, quantization=Round  (unbiased: +/- Inf), overflow=Wrap, coeffs_bit_limit=8, coeff_sharing=off, coeff_decimation=off, coeff_generation=off, cal_bits=1, n_bits_rotation=25, max_fanout=4, use_hdl=on, use_embedded=off, bitgrowth=off, hardcode_shifts=off, dsp48_adders=off}
      mask prompts: n_inputs "number inputs"; biplex "Used in biplex FFT"; FFTSize "Size of FFT: (2^? pts)"; Coeffs "Coefficients: (0 to 2^(FFTSize-1)-1)"; StepPeriod "Coefficient Step Period: (2^?)"; coeff_bit_width "Coefficient Bit Width"; input_bit_width "Input Bit Width"; bin_pt_in "Input binary point"; async "asynchronous operation"; floating_point "floating point"; float_type "float type"; exp_width "exponent width"; frac_width "fraction width"; add_latency "Add Latency"; mult_latency "Mult Latency"; bram_latency "BRAM Latency"; conv_latency "Convert latency"; add_pipe_latency "Add Pipeline Latency"; mult_pipe_latency "Mult Pipeline Latency"; quantization "Quantization Behavior"; overflow "Overflow Behavior"; coeffs_bit_limit "Number bits above which to store stage's coefficients in BRAM (2^? bits)"; coeff_sharing "BRAM sharing in coeff storage"; coeff_decimation "Store a fraction of coeff factors where useful"; coeff_generation "Generate coeffs with multipliers where useful"; cal_bits "Number calibration locations when generating coeffs (2^?)"; n_bits_rotation "Feedback rotation vector resolution"; max_fanout "Maximum fanout"; use_hdl "Use behavioural HDL for multipliers"; use_embedded "Use embedded multipliers"; bitgrowth "Bit growth instead of shifting"; hardcode_shifts "Hardcode shift schedule"; dsp48_adders "Use DSP48s for adders"
      mask help: FFT internal block.
      mask init: same as rfsoc4x2_ospfb_128/fft2/fft_direct/butterfly0_0
      settings: AttributesFormatString=twiddle_general
      mask Callback floating_point:
      | onoff = get_param(gcb, 'floating_point');
      | if strcmp(onoff,'on')
      |     enable_fixpt = 'off';
      |     set_param_state(gcb, 'float_type', 'on')
      | 
      |     f_type = get_param(gcb, 'float_type');
      |     if strcmp(f_type,'custom')
      |         set_param_state(gcb, 'exp_width', 'on')
      |         set_param_state(gcb, 'frac_width', 'on')
      |     else
      |         set_param_state(gcb, 'exp_width', 'off')
      |         set_param_state(gcb, 'frac_width', 'off')
      |     end
      | 
      | 
      | else
      |     enable_fixpt = 'on';
      |     set_param_state(gcb, 'float_type', 'off')
      |     set_param_state(gcb, 'exp_width', 'off')
      |     set_param_state(gcb, 'frac_width', 'off')
      | end
      | 
      | set_param_state(gcb, 'input_bit_width', enable_fixpt)
      | set_param_state(gcb, 'bin_pt_in', enable_fixpt)
      | set_param_state(gcb, 'coeff_bit_width', enable_fixpt)
      mask TypeOptions float_type: single | custom
      mask Callback float_type:
      | f_type = get_param(gcb, 'float_type');
      | if strcmp(f_type,'custom')
      |     set_param_state(gcb, 'exp_width', 'on')
      |     set_param_state(gcb, 'frac_width', 'on')
      | else
      |     set_param_state(gcb, 'exp_width', 'off')
      |     set_param_state(gcb, 'frac_width', 'off')
      | end
      mask TypeOptions quantization: Truncate | Round  (unbiased: +/- Inf) | Round  (unbiased: Even Values)
      mask TypeOptions overflow: Wrap | Saturate | Error
      mask Callback use_hdl:
      | % make mutually exclusive with use_embedded.
      | 
      | use_hdl = get_param(gcb, 'use_hdl');
      | if strcmp(use_hdl, 'on'),
      |     set_param_state(gcb, 'use_embedded', 'off');
      | else
      |     set_param_state(gcb, 'use_embedded', 'on');
      | end
      mask Callback use_embedded:
      | % make mutually exclusive with use_hdl.
      | 
      | use_hdl = get_param(gcb, 'use_embedded');
      | if strcmp(use_hdl, 'on'),
      |     set_param_state(gcb, 'use_hdl', 'off');
      | else
      |     set_param_state(gcb, 'use_hdl', 'on');
      | end
      mask Callback hardcode_shifts:
      | hardcode_shifts = get_param(gcb, 'hardcode_shifts');
      | set_param_state(gcb, 'downshift', hardcode_shifts);
      mask Callback dsp48_adders: %fft_callback_dsp48_adders(gcb);
      mask DialogControl ParameterTabVar0 Prompt: Basic
      mask DialogControl ParameterTabVar01 Prompt: Latency
      mask DialogControl ParameterTabVar012 Prompt: Implementation
  butterfly2_3 : Subsystem  AncestorBlock=casper_library_ffts/butterfly_direct  mask(butterfly_direct){n_inputs=2, biplex=off, FFTSize=8, Coeffs=[ 3 35 19 51 11 43 27 59 7 39 23 55 15 47 31 63], StepPeriod=0, coeff_bit_width=18, input_bit_width=18, bin_pt_in=17, downshift=off, async=off, floating_point=off, float_type=single, exp_width=8, frac_width=24, add_latency=1, mult_latency=3, bram_latency=3, conv_latency=3, add_pipe_latency=0, mult_pipe_latency=0, quantization=Round  (unbiased: +/- Inf), overflow=Wrap, coeffs_bit_limit=8, coeff_sharing=off, coeff_decimation=off, coeff_generation=off, cal_bits=1, n_bits_rotation=25, max_fanout=4, use_hdl=on, use_embedded=off, bitgrowth=off, hardcode_shifts=off, dsp48_adders=off}
      mask prompts: n_inputs "number inputs"; biplex "Used in biplex FFT"; FFTSize "Size of FFT: (2^? pts)"; Coeffs "Coefficients: (0 to 2^(FFTSize-1)-1)"; StepPeriod "Coefficient Step Period: (2^?)"; coeff_bit_width "Coefficient Bit Width"; input_bit_width "Input Bit Width"; bin_pt_in "Input binary point"; async "asynchronous operation"; floating_point "floating point"; float_type "float type"; exp_width "exponent width"; frac_width "fraction width"; add_latency "Add Latency"; mult_latency "Mult Latency"; bram_latency "BRAM Latency"; conv_latency "Convert latency"; add_pipe_latency "Add Pipeline Latency"; mult_pipe_latency "Mult Pipeline Latency"; quantization "Quantization Behavior"; overflow "Overflow Behavior"; coeffs_bit_limit "Number bits above which to store stage's coefficients in BRAM (2^? bits)"; coeff_sharing "BRAM sharing in coeff storage"; coeff_decimation "Store a fraction of coeff factors where useful"; coeff_generation "Generate coeffs with multipliers where useful"; cal_bits "Number calibration locations when generating coeffs (2^?)"; n_bits_rotation "Feedback rotation vector resolution"; max_fanout "Maximum fanout"; use_hdl "Use behavioural HDL for multipliers"; use_embedded "Use embedded multipliers"; bitgrowth "Bit growth instead of shifting"; hardcode_shifts "Hardcode shift schedule"; dsp48_adders "Use DSP48s for adders"
      mask help: FFT internal block.
      mask init: same as rfsoc4x2_ospfb_128/fft2/fft_direct/butterfly0_0
      settings: AttributesFormatString=twiddle_general
      mask Callback floating_point:
      | onoff = get_param(gcb, 'floating_point');
      | if strcmp(onoff,'on')
      |     enable_fixpt = 'off';
      |     set_param_state(gcb, 'float_type', 'on')
      | 
      |     f_type = get_param(gcb, 'float_type');
      |     if strcmp(f_type,'custom')
      |         set_param_state(gcb, 'exp_width', 'on')
      |         set_param_state(gcb, 'frac_width', 'on')
      |     else
      |         set_param_state(gcb, 'exp_width', 'off')
      |         set_param_state(gcb, 'frac_width', 'off')
      |     end
      | 
      | 
      | else
      |     enable_fixpt = 'on';
      |     set_param_state(gcb, 'float_type', 'off')
      |     set_param_state(gcb, 'exp_width', 'off')
      |     set_param_state(gcb, 'frac_width', 'off')
      | end
      | 
      | set_param_state(gcb, 'input_bit_width', enable_fixpt)
      | set_param_state(gcb, 'bin_pt_in', enable_fixpt)
      | set_param_state(gcb, 'coeff_bit_width', enable_fixpt)
      mask TypeOptions float_type: single | custom
      mask Callback float_type:
      | f_type = get_param(gcb, 'float_type');
      | if strcmp(f_type,'custom')
      |     set_param_state(gcb, 'exp_width', 'on')
      |     set_param_state(gcb, 'frac_width', 'on')
      | else
      |     set_param_state(gcb, 'exp_width', 'off')
      |     set_param_state(gcb, 'frac_width', 'off')
      | end
      mask TypeOptions quantization: Truncate | Round  (unbiased: +/- Inf) | Round  (unbiased: Even Values)
      mask TypeOptions overflow: Wrap | Saturate | Error
      mask Callback use_hdl:
      | % make mutually exclusive with use_embedded.
      | 
      | use_hdl = get_param(gcb, 'use_hdl');
      | if strcmp(use_hdl, 'on'),
      |     set_param_state(gcb, 'use_embedded', 'off');
      | else
      |     set_param_state(gcb, 'use_embedded', 'on');
      | end
      mask Callback use_embedded:
      | % make mutually exclusive with use_hdl.
      | 
      | use_hdl = get_param(gcb, 'use_embedded');
      | if strcmp(use_hdl, 'on'),
      |     set_param_state(gcb, 'use_hdl', 'off');
      | else
      |     set_param_state(gcb, 'use_hdl', 'on');
      | end
      mask Callback hardcode_shifts:
      | hardcode_shifts = get_param(gcb, 'hardcode_shifts');
      | set_param_state(gcb, 'downshift', hardcode_shifts);
      mask Callback dsp48_adders: %fft_callback_dsp48_adders(gcb);
      mask DialogControl ParameterTabVar0 Prompt: Basic
      mask DialogControl ParameterTabVar01 Prompt: Latency
      mask DialogControl ParameterTabVar012 Prompt: Implementation
  butterfly3_0 : Subsystem  AncestorBlock=casper_library_ffts/butterfly_direct  mask(butterfly_direct){n_inputs=1, biplex=off, FFTSize=8, Coeffs=[ 0 64 32 96 16 80 48 112 8 72 40 104 24 88 56 120], StepPeriod=0, coeff_bit_width=18, input_bit_width=18, bin_pt_in=17, downshift=off, async=off, floating_point=off, float_type=single, exp_width=8, frac_width=24, add_latency=1, mult_latency=3, bram_latency=3, conv_latency=3, add_pipe_latency=0, mult_pipe_latency=0, quantization=Round  (unbiased: +/- Inf), overflow=Wrap, coeffs_bit_limit=8, coeff_sharing=off, coeff_decimation=off, coeff_generation=off, cal_bits=1, n_bits_rotation=25, max_fanout=4, use_hdl=on, use_embedded=off, bitgrowth=off, hardcode_shifts=off, dsp48_adders=off}
      mask prompts: n_inputs "number inputs"; biplex "Used in biplex FFT"; FFTSize "Size of FFT: (2^? pts)"; Coeffs "Coefficients: (0 to 2^(FFTSize-1)-1)"; StepPeriod "Coefficient Step Period: (2^?)"; coeff_bit_width "Coefficient Bit Width"; input_bit_width "Input Bit Width"; bin_pt_in "Input binary point"; async "asynchronous operation"; floating_point "floating point"; float_type "float type"; exp_width "exponent width"; frac_width "fraction width"; add_latency "Add Latency"; mult_latency "Mult Latency"; bram_latency "BRAM Latency"; conv_latency "Convert latency"; add_pipe_latency "Add Pipeline Latency"; mult_pipe_latency "Mult Pipeline Latency"; quantization "Quantization Behavior"; overflow "Overflow Behavior"; coeffs_bit_limit "Number bits above which to store stage's coefficients in BRAM (2^? bits)"; coeff_sharing "BRAM sharing in coeff storage"; coeff_decimation "Store a fraction of coeff factors where useful"; coeff_generation "Generate coeffs with multipliers where useful"; cal_bits "Number calibration locations when generating coeffs (2^?)"; n_bits_rotation "Feedback rotation vector resolution"; max_fanout "Maximum fanout"; use_hdl "Use behavioural HDL for multipliers"; use_embedded "Use embedded multipliers"; bitgrowth "Bit growth instead of shifting"; hardcode_shifts "Hardcode shift schedule"; dsp48_adders "Use DSP48s for adders"
      mask help: FFT internal block.
      mask init: same as rfsoc4x2_ospfb_128/fft2/fft_direct/butterfly0_0
      settings: AttributesFormatString=twiddle_general
      mask Callback floating_point:
      | onoff = get_param(gcb, 'floating_point');
      | if strcmp(onoff,'on')
      |     enable_fixpt = 'off';
      |     set_param_state(gcb, 'float_type', 'on')
      | 
      |     f_type = get_param(gcb, 'float_type');
      |     if strcmp(f_type,'custom')
      |         set_param_state(gcb, 'exp_width', 'on')
      |         set_param_state(gcb, 'frac_width', 'on')
      |     else
      |         set_param_state(gcb, 'exp_width', 'off')
      |         set_param_state(gcb, 'frac_width', 'off')
      |     end
      | 
      | 
      | else
      |     enable_fixpt = 'on';
      |     set_param_state(gcb, 'float_type', 'off')
      |     set_param_state(gcb, 'exp_width', 'off')
      |     set_param_state(gcb, 'frac_width', 'off')
      | end
      | 
      | set_param_state(gcb, 'input_bit_width', enable_fixpt)
      | set_param_state(gcb, 'bin_pt_in', enable_fixpt)
      | set_param_state(gcb, 'coeff_bit_width', enable_fixpt)
      mask TypeOptions float_type: single | custom
      mask Callback float_type:
      | f_type = get_param(gcb, 'float_type');
      | if strcmp(f_type,'custom')
      |     set_param_state(gcb, 'exp_width', 'on')
      |     set_param_state(gcb, 'frac_width', 'on')
      | else
      |     set_param_state(gcb, 'exp_width', 'off')
      |     set_param_state(gcb, 'frac_width', 'off')
      | end
      mask TypeOptions quantization: Truncate | Round  (unbiased: +/- Inf) | Round  (unbiased: Even Values)
      mask TypeOptions overflow: Wrap | Saturate | Error
      mask Callback use_hdl:
      | % make mutually exclusive with use_embedded.
      | 
      | use_hdl = get_param(gcb, 'use_hdl');
      | if strcmp(use_hdl, 'on'),
      |     set_param_state(gcb, 'use_embedded', 'off');
      | else
      |     set_param_state(gcb, 'use_embedded', 'on');
      | end
      mask Callback use_embedded:
      | % make mutually exclusive with use_hdl.
      | 
      | use_hdl = get_param(gcb, 'use_embedded');
      | if strcmp(use_hdl, 'on'),
      |     set_param_state(gcb, 'use_hdl', 'off');
      | else
      |     set_param_state(gcb, 'use_hdl', 'on');
      | end
      mask Callback hardcode_shifts:
      | hardcode_shifts = get_param(gcb, 'hardcode_shifts');
      | set_param_state(gcb, 'downshift', hardcode_shifts);
      mask Callback dsp48_adders: %fft_callback_dsp48_adders(gcb);
      mask DialogControl ParameterTabVar0 Prompt: Basic
      mask DialogControl ParameterTabVar01 Prompt: Latency
      mask DialogControl ParameterTabVar012 Prompt: Implementation
  butterfly3_1 : Subsystem  AncestorBlock=casper_library_ffts/butterfly_direct  mask(butterfly_direct){n_inputs=1, biplex=off, FFTSize=8, Coeffs=[ 1 65 33 97 17 81 49 113 9 73 41 105 25 89 57 121], StepPeriod=0, coeff_bit_width=18, input_bit_width=18, bin_pt_in=17, downshift=off, async=off, floating_point=off, float_type=single, exp_width=8, frac_width=24, add_latency=1, mult_latency=3, bram_latency=3, conv_latency=3, add_pipe_latency=0, mult_pipe_latency=0, quantization=Round  (unbiased: +/- Inf), overflow=Wrap, coeffs_bit_limit=8, coeff_sharing=off, coeff_decimation=off, coeff_generation=off, cal_bits=1, n_bits_rotation=25, max_fanout=4, use_hdl=on, use_embedded=off, bitgrowth=off, hardcode_shifts=off, dsp48_adders=off}
      mask prompts: n_inputs "number inputs"; biplex "Used in biplex FFT"; FFTSize "Size of FFT: (2^? pts)"; Coeffs "Coefficients: (0 to 2^(FFTSize-1)-1)"; StepPeriod "Coefficient Step Period: (2^?)"; coeff_bit_width "Coefficient Bit Width"; input_bit_width "Input Bit Width"; bin_pt_in "Input binary point"; async "asynchronous operation"; floating_point "floating point"; float_type "float type"; exp_width "exponent width"; frac_width "fraction width"; add_latency "Add Latency"; mult_latency "Mult Latency"; bram_latency "BRAM Latency"; conv_latency "Convert latency"; add_pipe_latency "Add Pipeline Latency"; mult_pipe_latency "Mult Pipeline Latency"; quantization "Quantization Behavior"; overflow "Overflow Behavior"; coeffs_bit_limit "Number bits above which to store stage's coefficients in BRAM (2^? bits)"; coeff_sharing "BRAM sharing in coeff storage"; coeff_decimation "Store a fraction of coeff factors where useful"; coeff_generation "Generate coeffs with multipliers where useful"; cal_bits "Number calibration locations when generating coeffs (2^?)"; n_bits_rotation "Feedback rotation vector resolution"; max_fanout "Maximum fanout"; use_hdl "Use behavioural HDL for multipliers"; use_embedded "Use embedded multipliers"; bitgrowth "Bit growth instead of shifting"; hardcode_shifts "Hardcode shift schedule"; dsp48_adders "Use DSP48s for adders"
      mask help: FFT internal block.
      mask init: same as rfsoc4x2_ospfb_128/fft2/fft_direct/butterfly0_0
      settings: AttributesFormatString=twiddle_general
      mask Callback floating_point:
      | onoff = get_param(gcb, 'floating_point');
      | if strcmp(onoff,'on')
      |     enable_fixpt = 'off';
      |     set_param_state(gcb, 'float_type', 'on')
      | 
      |     f_type = get_param(gcb, 'float_type');
      |     if strcmp(f_type,'custom')
      |         set_param_state(gcb, 'exp_width', 'on')
      |         set_param_state(gcb, 'frac_width', 'on')
      |     else
      |         set_param_state(gcb, 'exp_width', 'off')
      |         set_param_state(gcb, 'frac_width', 'off')
      |     end
      | 
      | 
      | else
      |     enable_fixpt = 'on';
      |     set_param_state(gcb, 'float_type', 'off')
      |     set_param_state(gcb, 'exp_width', 'off')
      |     set_param_state(gcb, 'frac_width', 'off')
      | end
      | 
      | set_param_state(gcb, 'input_bit_width', enable_fixpt)
      | set_param_state(gcb, 'bin_pt_in', enable_fixpt)
      | set_param_state(gcb, 'coeff_bit_width', enable_fixpt)
      mask TypeOptions float_type: single | custom
      mask Callback float_type:
      | f_type = get_param(gcb, 'float_type');
      | if strcmp(f_type,'custom')
      |     set_param_state(gcb, 'exp_width', 'on')
      |     set_param_state(gcb, 'frac_width', 'on')
      | else
      |     set_param_state(gcb, 'exp_width', 'off')
      |     set_param_state(gcb, 'frac_width', 'off')
      | end
      mask TypeOptions quantization: Truncate | Round  (unbiased: +/- Inf) | Round  (unbiased: Even Values)
      mask TypeOptions overflow: Wrap | Saturate | Error
      mask Callback use_hdl:
      | % make mutually exclusive with use_embedded.
      | 
      | use_hdl = get_param(gcb, 'use_hdl');
      | if strcmp(use_hdl, 'on'),
      |     set_param_state(gcb, 'use_embedded', 'off');
      | else
      |     set_param_state(gcb, 'use_embedded', 'on');
      | end
      mask Callback use_embedded:
      | % make mutually exclusive with use_hdl.
      | 
      | use_hdl = get_param(gcb, 'use_embedded');
      | if strcmp(use_hdl, 'on'),
      |     set_param_state(gcb, 'use_hdl', 'off');
      | else
      |     set_param_state(gcb, 'use_hdl', 'on');
      | end
      mask Callback hardcode_shifts:
      | hardcode_shifts = get_param(gcb, 'hardcode_shifts');
      | set_param_state(gcb, 'downshift', hardcode_shifts);
      mask Callback dsp48_adders: %fft_callback_dsp48_adders(gcb);
      mask DialogControl ParameterTabVar0 Prompt: Basic
      mask DialogControl ParameterTabVar01 Prompt: Latency
      mask DialogControl ParameterTabVar012 Prompt: Implementation
  butterfly3_2 : Subsystem  AncestorBlock=casper_library_ffts/butterfly_direct  mask(butterfly_direct){n_inputs=1, biplex=off, FFTSize=8, Coeffs=[ 2 66 34 98 18 82 50 114 10 74 42 106 26 90 58 122], StepPeriod=0, coeff_bit_width=18, input_bit_width=18, bin_pt_in=17, downshift=off, async=off, floating_point=off, float_type=single, exp_width=8, frac_width=24, add_latency=1, mult_latency=3, bram_latency=3, conv_latency=3, add_pipe_latency=0, mult_pipe_latency=0, quantization=Round  (unbiased: +/- Inf), overflow=Wrap, coeffs_bit_limit=8, coeff_sharing=off, coeff_decimation=off, coeff_generation=off, cal_bits=1, n_bits_rotation=25, max_fanout=4, use_hdl=on, use_embedded=off, bitgrowth=off, hardcode_shifts=off, dsp48_adders=off}
      mask prompts: n_inputs "number inputs"; biplex "Used in biplex FFT"; FFTSize "Size of FFT: (2^? pts)"; Coeffs "Coefficients: (0 to 2^(FFTSize-1)-1)"; StepPeriod "Coefficient Step Period: (2^?)"; coeff_bit_width "Coefficient Bit Width"; input_bit_width "Input Bit Width"; bin_pt_in "Input binary point"; async "asynchronous operation"; floating_point "floating point"; float_type "float type"; exp_width "exponent width"; frac_width "fraction width"; add_latency "Add Latency"; mult_latency "Mult Latency"; bram_latency "BRAM Latency"; conv_latency "Convert latency"; add_pipe_latency "Add Pipeline Latency"; mult_pipe_latency "Mult Pipeline Latency"; quantization "Quantization Behavior"; overflow "Overflow Behavior"; coeffs_bit_limit "Number bits above which to store stage's coefficients in BRAM (2^? bits)"; coeff_sharing "BRAM sharing in coeff storage"; coeff_decimation "Store a fraction of coeff factors where useful"; coeff_generation "Generate coeffs with multipliers where useful"; cal_bits "Number calibration locations when generating coeffs (2^?)"; n_bits_rotation "Feedback rotation vector resolution"; max_fanout "Maximum fanout"; use_hdl "Use behavioural HDL for multipliers"; use_embedded "Use embedded multipliers"; bitgrowth "Bit growth instead of shifting"; hardcode_shifts "Hardcode shift schedule"; dsp48_adders "Use DSP48s for adders"
      mask help: FFT internal block.
      mask init: same as rfsoc4x2_ospfb_128/fft2/fft_direct/butterfly0_0
      settings: AttributesFormatString=twiddle_general
      mask Callback floating_point:
      | onoff = get_param(gcb, 'floating_point');
      | if strcmp(onoff,'on')
      |     enable_fixpt = 'off';
      |     set_param_state(gcb, 'float_type', 'on')
      | 
      |     f_type = get_param(gcb, 'float_type');
      |     if strcmp(f_type,'custom')
      |         set_param_state(gcb, 'exp_width', 'on')
      |         set_param_state(gcb, 'frac_width', 'on')
      |     else
      |         set_param_state(gcb, 'exp_width', 'off')
      |         set_param_state(gcb, 'frac_width', 'off')
      |     end
      | 
      | 
      | else
      |     enable_fixpt = 'on';
      |     set_param_state(gcb, 'float_type', 'off')
      |     set_param_state(gcb, 'exp_width', 'off')
      |     set_param_state(gcb, 'frac_width', 'off')
      | end
      | 
      | set_param_state(gcb, 'input_bit_width', enable_fixpt)
      | set_param_state(gcb, 'bin_pt_in', enable_fixpt)
      | set_param_state(gcb, 'coeff_bit_width', enable_fixpt)
      mask TypeOptions float_type: single | custom
      mask Callback float_type:
      | f_type = get_param(gcb, 'float_type');
      | if strcmp(f_type,'custom')
      |     set_param_state(gcb, 'exp_width', 'on')
      |     set_param_state(gcb, 'frac_width', 'on')
      | else
      |     set_param_state(gcb, 'exp_width', 'off')
      |     set_param_state(gcb, 'frac_width', 'off')
      | end
      mask TypeOptions quantization: Truncate | Round  (unbiased: +/- Inf) | Round  (unbiased: Even Values)
      mask TypeOptions overflow: Wrap | Saturate | Error
      mask Callback use_hdl:
      | % make mutually exclusive with use_embedded.
      | 
      | use_hdl = get_param(gcb, 'use_hdl');
      | if strcmp(use_hdl, 'on'),
      |     set_param_state(gcb, 'use_embedded', 'off');
      | else
      |     set_param_state(gcb, 'use_embedded', 'on');
      | end
      mask Callback use_embedded:
      | % make mutually exclusive with use_hdl.
      | 
      | use_hdl = get_param(gcb, 'use_embedded');
      | if strcmp(use_hdl, 'on'),
      |     set_param_state(gcb, 'use_hdl', 'off');
      | else
      |     set_param_state(gcb, 'use_hdl', 'on');
      | end
      mask Callback hardcode_shifts:
      | hardcode_shifts = get_param(gcb, 'hardcode_shifts');
      | set_param_state(gcb, 'downshift', hardcode_shifts);
      mask Callback dsp48_adders: %fft_callback_dsp48_adders(gcb);
      mask DialogControl ParameterTabVar0 Prompt: Basic
      mask DialogControl ParameterTabVar01 Prompt: Latency
      mask DialogControl ParameterTabVar012 Prompt: Implementation
  butterfly3_3 : Subsystem  AncestorBlock=casper_library_ffts/butterfly_direct  mask(butterfly_direct){n_inputs=1, biplex=off, FFTSize=8, Coeffs=[ 3 67 35 99 19 83 51 115 11 75 43 107 27 91 59 123], StepPeriod=0, coeff_bit_width=18, input_bit_width=18, bin_pt_in=17, downshift=off, async=off, floating_point=off, float_type=single, exp_width=8, frac_width=24, add_latency=1, mult_latency=3, bram_latency=3, conv_latency=3, add_pipe_latency=0, mult_pipe_latency=0, quantization=Round  (unbiased: +/- Inf), overflow=Wrap, coeffs_bit_limit=8, coeff_sharing=off, coeff_decimation=off, coeff_generation=off, cal_bits=1, n_bits_rotation=25, max_fanout=4, use_hdl=on, use_embedded=off, bitgrowth=off, hardcode_shifts=off, dsp48_adders=off}
      mask prompts: n_inputs "number inputs"; biplex "Used in biplex FFT"; FFTSize "Size of FFT: (2^? pts)"; Coeffs "Coefficients: (0 to 2^(FFTSize-1)-1)"; StepPeriod "Coefficient Step Period: (2^?)"; coeff_bit_width "Coefficient Bit Width"; input_bit_width "Input Bit Width"; bin_pt_in "Input binary point"; async "asynchronous operation"; floating_point "floating point"; float_type "float type"; exp_width "exponent width"; frac_width "fraction width"; add_latency "Add Latency"; mult_latency "Mult Latency"; bram_latency "BRAM Latency"; conv_latency "Convert latency"; add_pipe_latency "Add Pipeline Latency"; mult_pipe_latency "Mult Pipeline Latency"; quantization "Quantization Behavior"; overflow "Overflow Behavior"; coeffs_bit_limit "Number bits above which to store stage's coefficients in BRAM (2^? bits)"; coeff_sharing "BRAM sharing in coeff storage"; coeff_decimation "Store a fraction of coeff factors where useful"; coeff_generation "Generate coeffs with multipliers where useful"; cal_bits "Number calibration locations when generating coeffs (2^?)"; n_bits_rotation "Feedback rotation vector resolution"; max_fanout "Maximum fanout"; use_hdl "Use behavioural HDL for multipliers"; use_embedded "Use embedded multipliers"; bitgrowth "Bit growth instead of shifting"; hardcode_shifts "Hardcode shift schedule"; dsp48_adders "Use DSP48s for adders"
      mask help: FFT internal block.
      mask init: same as rfsoc4x2_ospfb_128/fft2/fft_direct/butterfly0_0
      settings: AttributesFormatString=twiddle_general
      mask Callback floating_point:
      | onoff = get_param(gcb, 'floating_point');
      | if strcmp(onoff,'on')
      |     enable_fixpt = 'off';
      |     set_param_state(gcb, 'float_type', 'on')
      | 
      |     f_type = get_param(gcb, 'float_type');
      |     if strcmp(f_type,'custom')
      |         set_param_state(gcb, 'exp_width', 'on')
      |         set_param_state(gcb, 'frac_width', 'on')
      |     else
      |         set_param_state(gcb, 'exp_width', 'off')
      |         set_param_state(gcb, 'frac_width', 'off')
      |     end
      | 
      | 
      | else
      |     enable_fixpt = 'on';
      |     set_param_state(gcb, 'float_type', 'off')
      |     set_param_state(gcb, 'exp_width', 'off')
      |     set_param_state(gcb, 'frac_width', 'off')
      | end
      | 
      | set_param_state(gcb, 'input_bit_width', enable_fixpt)
      | set_param_state(gcb, 'bin_pt_in', enable_fixpt)
      | set_param_state(gcb, 'coeff_bit_width', enable_fixpt)
      mask TypeOptions float_type: single | custom
      mask Callback float_type:
      | f_type = get_param(gcb, 'float_type');
      | if strcmp(f_type,'custom')
      |     set_param_state(gcb, 'exp_width', 'on')
      |     set_param_state(gcb, 'frac_width', 'on')
      | else
      |     set_param_state(gcb, 'exp_width', 'off')
      |     set_param_state(gcb, 'frac_width', 'off')
      | end
      mask TypeOptions quantization: Truncate | Round  (unbiased: +/- Inf) | Round  (unbiased: Even Values)
      mask TypeOptions overflow: Wrap | Saturate | Error
      mask Callback use_hdl:
      | % make mutually exclusive with use_embedded.
      | 
      | use_hdl = get_param(gcb, 'use_hdl');
      | if strcmp(use_hdl, 'on'),
      |     set_param_state(gcb, 'use_embedded', 'off');
      | else
      |     set_param_state(gcb, 'use_embedded', 'on');
      | end
      mask Callback use_embedded:
      | % make mutually exclusive with use_hdl.
      | 
      | use_hdl = get_param(gcb, 'use_embedded');
      | if strcmp(use_hdl, 'on'),
      |     set_param_state(gcb, 'use_hdl', 'off');
      | else
      |     set_param_state(gcb, 'use_hdl', 'on');
      | end
      mask Callback hardcode_shifts:
      | hardcode_shifts = get_param(gcb, 'hardcode_shifts');
      | set_param_state(gcb, 'downshift', hardcode_shifts);
      mask Callback dsp48_adders: %fft_callback_dsp48_adders(gcb);
      mask DialogControl ParameterTabVar0 Prompt: Basic
      mask DialogControl ParameterTabVar01 Prompt: Latency
      mask DialogControl ParameterTabVar012 Prompt: Implementation
  butterfly3_4 : Subsystem  AncestorBlock=casper_library_ffts/butterfly_direct  mask(butterfly_direct){n_inputs=1, biplex=off, FFTSize=8, Coeffs=[ 4 68 36 100 20 84 52 116 12 76 44 108 28 92 60 124], StepPeriod=0, coeff_bit_width=18, input_bit_width=18, bin_pt_in=17, downshift=off, async=off, floating_point=off, float_type=single, exp_width=8, frac_width=24, add_latency=1, mult_latency=3, bram_latency=3, conv_latency=3, add_pipe_latency=0, mult_pipe_latency=0, quantization=Round  (unbiased: +/- Inf), overflow=Wrap, coeffs_bit_limit=8, coeff_sharing=off, coeff_decimation=off, coeff_generation=off, cal_bits=1, n_bits_rotation=25, max_fanout=4, use_hdl=on, use_embedded=off, bitgrowth=off, hardcode_shifts=off, dsp48_adders=off}
      mask prompts: n_inputs "number inputs"; biplex "Used in biplex FFT"; FFTSize "Size of FFT: (2^? pts)"; Coeffs "Coefficients: (0 to 2^(FFTSize-1)-1)"; StepPeriod "Coefficient Step Period: (2^?)"; coeff_bit_width "Coefficient Bit Width"; input_bit_width "Input Bit Width"; bin_pt_in "Input binary point"; async "asynchronous operation"; floating_point "floating point"; float_type "float type"; exp_width "exponent width"; frac_width "fraction width"; add_latency "Add Latency"; mult_latency "Mult Latency"; bram_latency "BRAM Latency"; conv_latency "Convert latency"; add_pipe_latency "Add Pipeline Latency"; mult_pipe_latency "Mult Pipeline Latency"; quantization "Quantization Behavior"; overflow "Overflow Behavior"; coeffs_bit_limit "Number bits above which to store stage's coefficients in BRAM (2^? bits)"; coeff_sharing "BRAM sharing in coeff storage"; coeff_decimation "Store a fraction of coeff factors where useful"; coeff_generation "Generate coeffs with multipliers where useful"; cal_bits "Number calibration locations when generating coeffs (2^?)"; n_bits_rotation "Feedback rotation vector resolution"; max_fanout "Maximum fanout"; use_hdl "Use behavioural HDL for multipliers"; use_embedded "Use embedded multipliers"; bitgrowth "Bit growth instead of shifting"; hardcode_shifts "Hardcode shift schedule"; dsp48_adders "Use DSP48s for adders"
      mask help: FFT internal block.
      mask init: same as rfsoc4x2_ospfb_128/fft2/fft_direct/butterfly0_0
      settings: AttributesFormatString=twiddle_general
      mask Callback floating_point:
      | onoff = get_param(gcb, 'floating_point');
      | if strcmp(onoff,'on')
      |     enable_fixpt = 'off';
      |     set_param_state(gcb, 'float_type', 'on')
      | 
      |     f_type = get_param(gcb, 'float_type');
      |     if strcmp(f_type,'custom')
      |         set_param_state(gcb, 'exp_width', 'on')
      |         set_param_state(gcb, 'frac_width', 'on')
      |     else
      |         set_param_state(gcb, 'exp_width', 'off')
      |         set_param_state(gcb, 'frac_width', 'off')
      |     end
      | 
      | 
      | else
      |     enable_fixpt = 'on';
      |     set_param_state(gcb, 'float_type', 'off')
      |     set_param_state(gcb, 'exp_width', 'off')
      |     set_param_state(gcb, 'frac_width', 'off')
      | end
      | 
      | set_param_state(gcb, 'input_bit_width', enable_fixpt)
      | set_param_state(gcb, 'bin_pt_in', enable_fixpt)
      | set_param_state(gcb, 'coeff_bit_width', enable_fixpt)
      mask TypeOptions float_type: single | custom
      mask Callback float_type:
      | f_type = get_param(gcb, 'float_type');
      | if strcmp(f_type,'custom')
      |     set_param_state(gcb, 'exp_width', 'on')
      |     set_param_state(gcb, 'frac_width', 'on')
      | else
      |     set_param_state(gcb, 'exp_width', 'off')
      |     set_param_state(gcb, 'frac_width', 'off')
      | end
      mask TypeOptions quantization: Truncate | Round  (unbiased: +/- Inf) | Round  (unbiased: Even Values)
      mask TypeOptions overflow: Wrap | Saturate | Error
      mask Callback use_hdl:
      | % make mutually exclusive with use_embedded.
      | 
      | use_hdl = get_param(gcb, 'use_hdl');
      | if strcmp(use_hdl, 'on'),
      |     set_param_state(gcb, 'use_embedded', 'off');
      | else
      |     set_param_state(gcb, 'use_embedded', 'on');
      | end
      mask Callback use_embedded:
      | % make mutually exclusive with use_hdl.
      | 
      | use_hdl = get_param(gcb, 'use_embedded');
      | if strcmp(use_hdl, 'on'),
      |     set_param_state(gcb, 'use_hdl', 'off');
      | else
      |     set_param_state(gcb, 'use_hdl', 'on');
      | end
      mask Callback hardcode_shifts:
      | hardcode_shifts = get_param(gcb, 'hardcode_shifts');
      | set_param_state(gcb, 'downshift', hardcode_shifts);
      mask Callback dsp48_adders: %fft_callback_dsp48_adders(gcb);
      mask DialogControl ParameterTabVar0 Prompt: Basic
      mask DialogControl ParameterTabVar01 Prompt: Latency
      mask DialogControl ParameterTabVar012 Prompt: Implementation
  butterfly3_5 : Subsystem  AncestorBlock=casper_library_ffts/butterfly_direct  mask(butterfly_direct){n_inputs=1, biplex=off, FFTSize=8, Coeffs=[ 5 69 37 101 21 85 53 117 13 77 45 109 29 93 61 125], StepPeriod=0, coeff_bit_width=18, input_bit_width=18, bin_pt_in=17, downshift=off, async=off, floating_point=off, float_type=single, exp_width=8, frac_width=24, add_latency=1, mult_latency=3, bram_latency=3, conv_latency=3, add_pipe_latency=0, mult_pipe_latency=0, quantization=Round  (unbiased: +/- Inf), overflow=Wrap, coeffs_bit_limit=8, coeff_sharing=off, coeff_decimation=off, coeff_generation=off, cal_bits=1, n_bits_rotation=25, max_fanout=4, use_hdl=on, use_embedded=off, bitgrowth=off, hardcode_shifts=off, dsp48_adders=off}
      mask prompts: n_inputs "number inputs"; biplex "Used in biplex FFT"; FFTSize "Size of FFT: (2^? pts)"; Coeffs "Coefficients: (0 to 2^(FFTSize-1)-1)"; StepPeriod "Coefficient Step Period: (2^?)"; coeff_bit_width "Coefficient Bit Width"; input_bit_width "Input Bit Width"; bin_pt_in "Input binary point"; async "asynchronous operation"; floating_point "floating point"; float_type "float type"; exp_width "exponent width"; frac_width "fraction width"; add_latency "Add Latency"; mult_latency "Mult Latency"; bram_latency "BRAM Latency"; conv_latency "Convert latency"; add_pipe_latency "Add Pipeline Latency"; mult_pipe_latency "Mult Pipeline Latency"; quantization "Quantization Behavior"; overflow "Overflow Behavior"; coeffs_bit_limit "Number bits above which to store stage's coefficients in BRAM (2^? bits)"; coeff_sharing "BRAM sharing in coeff storage"; coeff_decimation "Store a fraction of coeff factors where useful"; coeff_generation "Generate coeffs with multipliers where useful"; cal_bits "Number calibration locations when generating coeffs (2^?)"; n_bits_rotation "Feedback rotation vector resolution"; max_fanout "Maximum fanout"; use_hdl "Use behavioural HDL for multipliers"; use_embedded "Use embedded multipliers"; bitgrowth "Bit growth instead of shifting"; hardcode_shifts "Hardcode shift schedule"; dsp48_adders "Use DSP48s for adders"
      mask help: FFT internal block.
      mask init: same as rfsoc4x2_ospfb_128/fft2/fft_direct/butterfly0_0
      settings: AttributesFormatString=twiddle_general
      mask Callback floating_point:
      | onoff = get_param(gcb, 'floating_point');
      | if strcmp(onoff,'on')
      |     enable_fixpt = 'off';
      |     set_param_state(gcb, 'float_type', 'on')
      | 
      |     f_type = get_param(gcb, 'float_type');
      |     if strcmp(f_type,'custom')
      |         set_param_state(gcb, 'exp_width', 'on')
      |         set_param_state(gcb, 'frac_width', 'on')
      |     else
      |         set_param_state(gcb, 'exp_width', 'off')
      |         set_param_state(gcb, 'frac_width', 'off')
      |     end
      | 
      | 
      | else
      |     enable_fixpt = 'on';
      |     set_param_state(gcb, 'float_type', 'off')
      |     set_param_state(gcb, 'exp_width', 'off')
      |     set_param_state(gcb, 'frac_width', 'off')
      | end
      | 
      | set_param_state(gcb, 'input_bit_width', enable_fixpt)
      | set_param_state(gcb, 'bin_pt_in', enable_fixpt)
      | set_param_state(gcb, 'coeff_bit_width', enable_fixpt)
      mask TypeOptions float_type: single | custom
      mask Callback float_type:
      | f_type = get_param(gcb, 'float_type');
      | if strcmp(f_type,'custom')
      |     set_param_state(gcb, 'exp_width', 'on')
      |     set_param_state(gcb, 'frac_width', 'on')
      | else
      |     set_param_state(gcb, 'exp_width', 'off')
      |     set_param_state(gcb, 'frac_width', 'off')
      | end
      mask TypeOptions quantization: Truncate | Round  (unbiased: +/- Inf) | Round  (unbiased: Even Values)
      mask TypeOptions overflow: Wrap | Saturate | Error
      mask Callback use_hdl:
      | % make mutually exclusive with use_embedded.
      | 
      | use_hdl = get_param(gcb, 'use_hdl');
      | if strcmp(use_hdl, 'on'),
      |     set_param_state(gcb, 'use_embedded', 'off');
      | else
      |     set_param_state(gcb, 'use_embedded', 'on');
      | end
      mask Callback use_embedded:
      | % make mutually exclusive with use_hdl.
      | 
      | use_hdl = get_param(gcb, 'use_embedded');
      | if strcmp(use_hdl, 'on'),
      |     set_param_state(gcb, 'use_hdl', 'off');
      | else
      |     set_param_state(gcb, 'use_hdl', 'on');
      | end
      mask Callback hardcode_shifts:
      | hardcode_shifts = get_param(gcb, 'hardcode_shifts');
      | set_param_state(gcb, 'downshift', hardcode_shifts);
      mask Callback dsp48_adders: %fft_callback_dsp48_adders(gcb);
      mask DialogControl ParameterTabVar0 Prompt: Basic
      mask DialogControl ParameterTabVar01 Prompt: Latency
      mask DialogControl ParameterTabVar012 Prompt: Implementation
  butterfly3_6 : Subsystem  AncestorBlock=casper_library_ffts/butterfly_direct  mask(butterfly_direct){n_inputs=1, biplex=off, FFTSize=8, Coeffs=[ 6 70 38 102 22 86 54 118 14 78 46 110 30 94 62 126], StepPeriod=0, coeff_bit_width=18, input_bit_width=18, bin_pt_in=17, downshift=off, async=off, floating_point=off, float_type=single, exp_width=8, frac_width=24, add_latency=1, mult_latency=3, bram_latency=3, conv_latency=3, add_pipe_latency=0, mult_pipe_latency=0, quantization=Round  (unbiased: +/- Inf), overflow=Wrap, coeffs_bit_limit=8, coeff_sharing=off, coeff_decimation=off, coeff_generation=off, cal_bits=1, n_bits_rotation=25, max_fanout=4, use_hdl=on, use_embedded=off, bitgrowth=off, hardcode_shifts=off, dsp48_adders=off}
      mask prompts: n_inputs "number inputs"; biplex "Used in biplex FFT"; FFTSize "Size of FFT: (2^? pts)"; Coeffs "Coefficients: (0 to 2^(FFTSize-1)-1)"; StepPeriod "Coefficient Step Period: (2^?)"; coeff_bit_width "Coefficient Bit Width"; input_bit_width "Input Bit Width"; bin_pt_in "Input binary point"; async "asynchronous operation"; floating_point "floating point"; float_type "float type"; exp_width "exponent width"; frac_width "fraction width"; add_latency "Add Latency"; mult_latency "Mult Latency"; bram_latency "BRAM Latency"; conv_latency "Convert latency"; add_pipe_latency "Add Pipeline Latency"; mult_pipe_latency "Mult Pipeline Latency"; quantization "Quantization Behavior"; overflow "Overflow Behavior"; coeffs_bit_limit "Number bits above which to store stage's coefficients in BRAM (2^? bits)"; coeff_sharing "BRAM sharing in coeff storage"; coeff_decimation "Store a fraction of coeff factors where useful"; coeff_generation "Generate coeffs with multipliers where useful"; cal_bits "Number calibration locations when generating coeffs (2^?)"; n_bits_rotation "Feedback rotation vector resolution"; max_fanout "Maximum fanout"; use_hdl "Use behavioural HDL for multipliers"; use_embedded "Use embedded multipliers"; bitgrowth "Bit growth instead of shifting"; hardcode_shifts "Hardcode shift schedule"; dsp48_adders "Use DSP48s for adders"
      mask help: FFT internal block.
      mask init: same as rfsoc4x2_ospfb_128/fft2/fft_direct/butterfly0_0
      settings: AttributesFormatString=twiddle_general
      mask Callback floating_point:
      | onoff = get_param(gcb, 'floating_point');
      | if strcmp(onoff,'on')
      |     enable_fixpt = 'off';
      |     set_param_state(gcb, 'float_type', 'on')
      | 
      |     f_type = get_param(gcb, 'float_type');
      |     if strcmp(f_type,'custom')
      |         set_param_state(gcb, 'exp_width', 'on')
      |         set_param_state(gcb, 'frac_width', 'on')
      |     else
      |         set_param_state(gcb, 'exp_width', 'off')
      |         set_param_state(gcb, 'frac_width', 'off')
      |     end
      | 
      | 
      | else
      |     enable_fixpt = 'on';
      |     set_param_state(gcb, 'float_type', 'off')
      |     set_param_state(gcb, 'exp_width', 'off')
      |     set_param_state(gcb, 'frac_width', 'off')
      | end
      | 
      | set_param_state(gcb, 'input_bit_width', enable_fixpt)
      | set_param_state(gcb, 'bin_pt_in', enable_fixpt)
      | set_param_state(gcb, 'coeff_bit_width', enable_fixpt)
      mask TypeOptions float_type: single | custom
      mask Callback float_type:
      | f_type = get_param(gcb, 'float_type');
      | if strcmp(f_type,'custom')
      |     set_param_state(gcb, 'exp_width', 'on')
      |     set_param_state(gcb, 'frac_width', 'on')
      | else
      |     set_param_state(gcb, 'exp_width', 'off')
      |     set_param_state(gcb, 'frac_width', 'off')
      | end
      mask TypeOptions quantization: Truncate | Round  (unbiased: +/- Inf) | Round  (unbiased: Even Values)
      mask TypeOptions overflow: Wrap | Saturate | Error
      mask Callback use_hdl:
      | % make mutually exclusive with use_embedded.
      | 
      | use_hdl = get_param(gcb, 'use_hdl');
      | if strcmp(use_hdl, 'on'),
      |     set_param_state(gcb, 'use_embedded', 'off');
      | else
      |     set_param_state(gcb, 'use_embedded', 'on');
      | end
      mask Callback use_embedded:
      | % make mutually exclusive with use_hdl.
      | 
      | use_hdl = get_param(gcb, 'use_embedded');
      | if strcmp(use_hdl, 'on'),
      |     set_param_state(gcb, 'use_hdl', 'off');
      | else
      |     set_param_state(gcb, 'use_hdl', 'on');
      | end
      mask Callback hardcode_shifts:
      | hardcode_shifts = get_param(gcb, 'hardcode_shifts');
      | set_param_state(gcb, 'downshift', hardcode_shifts);
      mask Callback dsp48_adders: %fft_callback_dsp48_adders(gcb);
      mask DialogControl ParameterTabVar0 Prompt: Basic
      mask DialogControl ParameterTabVar01 Prompt: Latency
      mask DialogControl ParameterTabVar012 Prompt: Implementation
  butterfly3_7 : Subsystem  AncestorBlock=casper_library_ffts/butterfly_direct  mask(butterfly_direct){n_inputs=1, biplex=off, FFTSize=8, Coeffs=[ 7 71 39 103 23 87 55 119 15 79 47 111 31 95 63 127], StepPeriod=0, coeff_bit_width=18, input_bit_width=18, bin_pt_in=17, downshift=off, async=off, floating_point=off, float_type=single, exp_width=8, frac_width=24, add_latency=1, mult_latency=3, bram_latency=3, conv_latency=3, add_pipe_latency=0, mult_pipe_latency=0, quantization=Round  (unbiased: +/- Inf), overflow=Wrap, coeffs_bit_limit=8, coeff_sharing=off, coeff_decimation=off, coeff_generation=off, cal_bits=1, n_bits_rotation=25, max_fanout=4, use_hdl=on, use_embedded=off, bitgrowth=off, hardcode_shifts=off, dsp48_adders=off}
      mask prompts: n_inputs "number inputs"; biplex "Used in biplex FFT"; FFTSize "Size of FFT: (2^? pts)"; Coeffs "Coefficients: (0 to 2^(FFTSize-1)-1)"; StepPeriod "Coefficient Step Period: (2^?)"; coeff_bit_width "Coefficient Bit Width"; input_bit_width "Input Bit Width"; bin_pt_in "Input binary point"; async "asynchronous operation"; floating_point "floating point"; float_type "float type"; exp_width "exponent width"; frac_width "fraction width"; add_latency "Add Latency"; mult_latency "Mult Latency"; bram_latency "BRAM Latency"; conv_latency "Convert latency"; add_pipe_latency "Add Pipeline Latency"; mult_pipe_latency "Mult Pipeline Latency"; quantization "Quantization Behavior"; overflow "Overflow Behavior"; coeffs_bit_limit "Number bits above which to store stage's coefficients in BRAM (2^? bits)"; coeff_sharing "BRAM sharing in coeff storage"; coeff_decimation "Store a fraction of coeff factors where useful"; coeff_generation "Generate coeffs with multipliers where useful"; cal_bits "Number calibration locations when generating coeffs (2^?)"; n_bits_rotation "Feedback rotation vector resolution"; max_fanout "Maximum fanout"; use_hdl "Use behavioural HDL for multipliers"; use_embedded "Use embedded multipliers"; bitgrowth "Bit growth instead of shifting"; hardcode_shifts "Hardcode shift schedule"; dsp48_adders "Use DSP48s for adders"
      mask help: FFT internal block.
      mask init: same as rfsoc4x2_ospfb_128/fft2/fft_direct/butterfly0_0
      settings: AttributesFormatString=twiddle_general
      mask Callback floating_point:
      | onoff = get_param(gcb, 'floating_point');
      | if strcmp(onoff,'on')
      |     enable_fixpt = 'off';
      |     set_param_state(gcb, 'float_type', 'on')
      | 
      |     f_type = get_param(gcb, 'float_type');
      |     if strcmp(f_type,'custom')
      |         set_param_state(gcb, 'exp_width', 'on')
      |         set_param_state(gcb, 'frac_width', 'on')
      |     else
      |         set_param_state(gcb, 'exp_width', 'off')
      |         set_param_state(gcb, 'frac_width', 'off')
      |     end
      | 
      | 
      | else
      |     enable_fixpt = 'on';
      |     set_param_state(gcb, 'float_type', 'off')
      |     set_param_state(gcb, 'exp_width', 'off')
      |     set_param_state(gcb, 'frac_width', 'off')
      | end
      | 
      | set_param_state(gcb, 'input_bit_width', enable_fixpt)
      | set_param_state(gcb, 'bin_pt_in', enable_fixpt)
      | set_param_state(gcb, 'coeff_bit_width', enable_fixpt)
      mask TypeOptions float_type: single | custom
      mask Callback float_type:
      | f_type = get_param(gcb, 'float_type');
      | if strcmp(f_type,'custom')
      |     set_param_state(gcb, 'exp_width', 'on')
      |     set_param_state(gcb, 'frac_width', 'on')
      | else
      |     set_param_state(gcb, 'exp_width', 'off')
      |     set_param_state(gcb, 'frac_width', 'off')
      | end
      mask TypeOptions quantization: Truncate | Round  (unbiased: +/- Inf) | Round  (unbiased: Even Values)
      mask TypeOptions overflow: Wrap | Saturate | Error
      mask Callback use_hdl:
      | % make mutually exclusive with use_embedded.
      | 
      | use_hdl = get_param(gcb, 'use_hdl');
      | if strcmp(use_hdl, 'on'),
      |     set_param_state(gcb, 'use_embedded', 'off');
      | else
      |     set_param_state(gcb, 'use_embedded', 'on');
      | end
      mask Callback use_embedded:
      | % make mutually exclusive with use_hdl.
      | 
      | use_hdl = get_param(gcb, 'use_embedded');
      | if strcmp(use_hdl, 'on'),
      |     set_param_state(gcb, 'use_hdl', 'off');
      | else
      |     set_param_state(gcb, 'use_hdl', 'on');
      | end
      mask Callback hardcode_shifts:
      | hardcode_shifts = get_param(gcb, 'hardcode_shifts');
      | set_param_state(gcb, 'downshift', hardcode_shifts);
      mask Callback dsp48_adders: %fft_callback_dsp48_adders(gcb);
      mask DialogControl ParameterTabVar0 Prompt: Basic
      mask DialogControl ParameterTabVar01 Prompt: Latency
      mask DialogControl ParameterTabVar012 Prompt: Implementation
  combine : xbsIndex_r4/Logical  logical_function=OR  inputs=8  en=off  latency=2  precision=Full  arith_type=Unsigned  n_bits=16  bin_pt=0  align_bp=on  dbl_ovrd=off  block_type=logical
  of_0 : xbsIndex_r4/Delay  rst=off  infoeditControl=Selection of Reset will increase slice count due to use of real FFs and instead of SRLs  en=off  latency=0  reg_retiming=on  dbl_ovrd=off  block_type=delay
  of_1 : xbsIndex_r4/Concat  num_inputs=2  dbl_ovrd=off  block_type=concat
  of_2 : xbsIndex_r4/Concat  num_inputs=4  dbl_ovrd=off  block_type=concat
  of_3 : xbsIndex_r4/Concat  num_inputs=8  dbl_ovrd=off  block_type=concat
  of_expand : Subsystem  AncestorBlock=casper_library_flow_control/bus_expand  mask(bus_expand){mode=divisions of equal size, outputNum=8, outputWidth=1, outputBinaryPt=0, outputArithmeticType=0, show_format=off, outputToWorkspace=off, variablePrefix=out, outputToModelAsWell=on}
      mask prompts: outputNum "Number of outputs:"; outputWidth "Output width:"; outputBinaryPt "Output binary point position:"; outputArithmeticType "Output arithmetic type (ufix=0, fix=1, bool=2):"; show_format "Print format string?"; outputToWorkspace "Output to workspace?"; variablePrefix "Variable name prefix:"; outputToModelAsWell "Output to model as well?"
      mask help:
      | Expands a 'bus' made using a bus_create or Xilinx
      | concat block.
      | The input will be divided into the specified number
      | of outputs with the specified arithmetic types.
      | Divisions are made from most significant bit.
      mask init: same as rfsoc4x2_ospfb_128/bus_expand1
      settings: AttributesFormatString=8 outputs
      mask TypeOptions mode: divisions of equal size | divisions of arbitrary size
      mask Callback mode: %bus_expand_callback();
      mask Callback outputWidth: %bus_expand_callback();
      mask Callback outputToWorkspace: %bus_expand_callback();
  of_or : xbsIndex_r4/Logical  logical_function=OR  inputs=4  en=off  latency=2  precision=Full  arith_type=Unsigned  n_bits=16  bin_pt=0  align_bp=on  dbl_ovrd=off  block_type=logical
  slice0 : xbsIndex_r4/Slice  nbits=1  boolean_output=on  mode=Lower Bit Location + Width  bit1=0  base1=MSB of Input  bit0=0  base0=LSB of Input  dbl_ovrd=off  block_type=slice
  slice1 : xbsIndex_r4/Slice  nbits=1  boolean_output=on  mode=Lower Bit Location + Width  bit1=0  base1=MSB of Input  bit0=1  base0=LSB of Input  dbl_ovrd=off  block_type=slice
  slice2 : xbsIndex_r4/Slice  nbits=1  boolean_output=on  mode=Lower Bit Location + Width  bit1=0  base1=MSB of Input  bit0=2  base0=LSB of Input  dbl_ovrd=off  block_type=slice
  slice3 : xbsIndex_r4/Slice  nbits=1  boolean_output=on  mode=Lower Bit Location + Width  bit1=0  base1=MSB of Input  bit0=3  base0=LSB of Input  dbl_ovrd=off  block_type=slice
  synct{1..7} (7 alike) : Terminator
  sync_out : Outport
  out00 : Outport  Port=2
  out01 : Outport  Port=3
  out02 : Outport  Port=4
  out03 : Outport  Port=5
  out04 : Outport  Port=6
  out05 : Outport  Port=7
  out06 : Outport  Port=8
  out07 : Outport  Port=9
  out08 : Outport  Port=10
  out09 : Outport  Port=11
  out010 : Outport  Port=12
  out011 : Outport  Port=13
  out012 : Outport  Port=14
  out013 : Outport  Port=15
  out014 : Outport  Port=16
  out015 : Outport  Port=17
  of : Outport  Port=18
  wires:
  butterfly3_7/2(a-bw) -> bdebus3_7/1(bus_in)
  butterfly3_7/1(a+bw) -> adebus3_7/1(bus_in)
  butterfly3_6/2(a-bw) -> bdebus3_6/1(bus_in)
  butterfly3_6/1(a+bw) -> adebus3_6/1(bus_in)
  butterfly3_5/2(a-bw) -> bdebus3_5/1(bus_in)
  butterfly3_5/1(a+bw) -> adebus3_5/1(bus_in)
  butterfly3_4/2(a-bw) -> bdebus3_4/1(bus_in)
  butterfly3_4/1(a+bw) -> adebus3_4/1(bus_in)
  butterfly3_3/2(a-bw) -> bdebus3_3/1(bus_in)
  butterfly3_3/1(a+bw) -> adebus3_3/1(bus_in)
  butterfly3_2/2(a-bw) -> bdebus3_2/1(bus_in)
  butterfly3_2/1(a+bw) -> adebus3_2/1(bus_in)
  butterfly3_1/2(a-bw) -> bdebus3_1/1(bus_in)
  butterfly3_1/1(a+bw) -> adebus3_1/1(bus_in)
  butterfly3_0/2(a-bw) -> bdebus3_0/1(bus_in)
  butterfly3_0/1(a+bw) -> adebus3_0/1(bus_in)
  butterfly3_7/3(of) -> of_3/8
  bdebus2_3/2(lsb_out1) -> butterfly3_7/2(b)
  bdebus2_3/1(msb_out2) -> butterfly3_7/1(a)
  butterfly3_7/4(sync_out) -> synct7/1
  butterfly3_6/3(of) -> of_3/7
  adebus2_3/2(lsb_out1) -> butterfly3_6/2(b)
  adebus2_3/1(msb_out2) -> butterfly3_6/1(a)
  butterfly3_6/4(sync_out) -> synct6/1
  butterfly2_3/4(sync_out) -> butterfly3_7/3(sync_in), butterfly3_6/3(sync_in)
  butterfly3_5/3(of) -> of_3/6
  bdebus2_2/2(lsb_out1) -> butterfly3_5/2(b)
  bdebus2_2/1(msb_out2) -> butterfly3_5/1(a)
  butterfly3_5/4(sync_out) -> synct5/1
  butterfly3_4/3(of) -> of_3/5
  adebus2_2/2(lsb_out1) -> butterfly3_4/2(b)
  adebus2_2/1(msb_out2) -> butterfly3_4/1(a)
  butterfly3_4/4(sync_out) -> synct4/1
  butterfly2_2/4(sync_out) -> butterfly3_5/3(sync_in), butterfly3_4/3(sync_in)
  butterfly3_3/3(of) -> of_3/4
  bdebus2_1/2(lsb_out1) -> butterfly3_3/2(b)
  bdebus2_1/1(msb_out2) -> butterfly3_3/1(a)
  butterfly3_3/4(sync_out) -> synct3/1
  butterfly3_2/3(of) -> of_3/3
  adebus2_1/2(lsb_out1) -> butterfly3_2/2(b)
  adebus2_1/1(msb_out2) -> butterfly3_2/1(a)
  butterfly3_2/4(sync_out) -> synct2/1
  butterfly2_1/4(sync_out) -> butterfly3_3/3(sync_in), butterfly3_2/3(sync_in)
  butterfly3_1/3(of) -> of_3/2
  bdebus2_0/2(lsb_out1) -> butterfly3_1/2(b)
  bdebus2_0/1(msb_out2) -> butterfly3_1/1(a)
  butterfly3_1/4(sync_out) -> synct1/1
  butterfly3_0/3(of) -> of_3/1
  adebus2_0/2(lsb_out1) -> butterfly3_0/2(b)
  adebus2_0/1(msb_out2) -> butterfly3_0/1(a)
  slice3/1 -> butterfly3_7/4(shift), butterfly3_6/4(shift), butterfly3_5/4(shift), butterfly3_4/4(shift), butterfly3_3/4(shift), butterfly3_2/4(shift), butterfly3_1/4(shift), butterfly3_0/4(shift)
  butterfly3_0/4(sync_out) -> sync_out/1
  butterfly2_0/4(sync_out) -> butterfly3_1/3(sync_in), butterfly3_0/3(sync_in)
  of_3/1 -> of_or/4
  butterfly2_3/2(a-bw) -> bdebus2_3/1(bus_in)
  butterfly2_3/1(a+bw) -> adebus2_3/1(bus_in)
  butterfly2_3/3(of) -> of_2/4
  bdebus1_1/2(lsb_out1) -> butterfly2_3/2(b)
  bdebus1_1/1(msb_out2) -> butterfly2_3/1(a)
  butterfly2_2/2(a-bw) -> bdebus2_2/1(bus_in)
  butterfly2_2/1(a+bw) -> adebus2_2/1(bus_in)
  butterfly2_2/3(of) -> of_2/3
  adebus1_1/2(lsb_out1) -> butterfly2_2/2(b)
  adebus1_1/1(msb_out2) -> butterfly2_2/1(a)
  butterfly1_1/4(sync_out) -> butterfly2_3/3(sync_in), butterfly2_2/3(sync_in)
  butterfly2_1/2(a-bw) -> bdebus2_1/1(bus_in)
  butterfly2_1/1(a+bw) -> adebus2_1/1(bus_in)
  butterfly2_1/3(of) -> of_2/2
  bdebus1_0/2(lsb_out1) -> butterfly2_1/2(b)
  bdebus1_0/1(msb_out2) -> butterfly2_1/1(a)
  butterfly2_0/2(a-bw) -> bdebus2_0/1(bus_in)
  butterfly2_0/1(a+bw) -> adebus2_0/1(bus_in)
  butterfly2_0/3(of) -> of_2/1
  adebus1_0/2(lsb_out1) -> butterfly2_0/2(b)
  adebus1_0/1(msb_out2) -> butterfly2_0/1(a)
  slice2/1 -> butterfly2_3/4(shift), butterfly2_2/4(shift), butterfly2_1/4(shift), butterfly2_0/4(shift)
  butterfly1_0/4(sync_out) -> butterfly2_1/3(sync_in), butterfly2_0/3(sync_in)
  of_2/1 -> of_or/3
  butterfly1_1/2(a-bw) -> bdebus1_1/1(bus_in)
  butterfly1_1/1(a+bw) -> adebus1_1/1(bus_in)
  butterfly1_1/3(of) -> of_1/2
  bdebus0_0/2(lsb_out1) -> butterfly1_1/2(b)
  bdebus0_0/1(msb_out2) -> butterfly1_1/1(a)
  butterfly1_0/2(a-bw) -> bdebus1_0/1(bus_in)
  butterfly1_0/1(a+bw) -> adebus1_0/1(bus_in)
  butterfly1_0/3(of) -> of_1/1
  adebus0_0/2(lsb_out1) -> butterfly1_0/2(b)
  adebus0_0/1(msb_out2) -> butterfly1_0/1(a)
  slice1/1 -> butterfly1_1/4(shift), butterfly1_0/4(shift)
  butterfly0_0/4(sync_out) -> butterfly1_1/3(sync_in), butterfly1_0/3(sync_in)
  of_1/1 -> of_or/2
  butterfly0_0/2(a-bw) -> bdebus0_0/1(bus_in)
  butterfly0_0/1(a+bw) -> adebus0_0/1(bus_in)
  butterfly0_0/3(of) -> of_0/1
  bbus/1(bus_out) -> butterfly0_0/2(b)
  abus/1(bus_out) -> butterfly0_0/1(a)
  slice0/1 -> butterfly0_0/4(shift)
  sync/1 -> butterfly0_0/3(sync_in)
  of_0/1 -> of_or/1
  shift/1 -> slice3/1, slice2/1, slice1/1, slice0/1
  combine/1 -> of/1
  of_expand/8(lsb_out1) -> combine/8
  of_expand/7(out2) -> combine/7
  of_expand/6(out3) -> combine/6
  of_expand/5(out4) -> combine/5
  of_expand/4(out5) -> combine/4
  of_expand/3(out6) -> combine/3
  of_expand/2(out7) -> combine/2
  of_expand/1(msb_out8) -> combine/1
  of_or/1 -> of_expand/1(bus_in)
  bdebus3_7/1(msb_lsb_out1) -> out015/1
  in015/1 -> bbus/8(in8)
  bdebus3_3/1(msb_lsb_out1) -> out014/1
  in014/1 -> bbus/7(in7)
  bdebus3_5/1(msb_lsb_out1) -> out013/1
  in013/1 -> bbus/6(in6)
  bdebus3_1/1(msb_lsb_out1) -> out012/1
  in012/1 -> bbus/5(in5)
  bdebus3_6/1(msb_lsb_out1) -> out011/1
  in011/1 -> bbus/4(in4)
  bdebus3_2/1(msb_lsb_out1) -> out010/1
  in010/1 -> bbus/3(in3)
  bdebus3_4/1(msb_lsb_out1) -> out09/1
  in09/1 -> bbus/2(in2)
  bdebus3_0/1(msb_lsb_out1) -> out08/1
  in08/1 -> bbus/1(in1)
  adebus3_7/1(msb_lsb_out1) -> out07/1
  in07/1 -> abus/8(in8)
  adebus3_3/1(msb_lsb_out1) -> out06/1
  in06/1 -> abus/7(in7)
  adebus3_5/1(msb_lsb_out1) -> out05/1
  in05/1 -> abus/6(in6)
  adebus3_1/1(msb_lsb_out1) -> out04/1
  in04/1 -> abus/5(in5)
  adebus3_6/1(msb_lsb_out1) -> out03/1
  in03/1 -> abus/4(in4)
  adebus3_2/1(msb_lsb_out1) -> out02/1
  in02/1 -> abus/3(in3)
  adebus3_4/1(msb_lsb_out1) -> out01/1
  in01/1 -> abus/2(in2)
  adebus3_0/1(msb_lsb_out1) -> out00/1
  in00/1 -> abus/1(in1)
